simulink model "FullFMS_2026_02_18_V0_3_9"  (R2025b)
settings: Solver=ode23tb  StartTime=0.0  StopTime=inf  MaxStep=0.1  RelTol=1e-2
PreLoadFcn:
  | load("BUS_CONFIG.mat")
libraries: opcualib x8
(part 3 of 4)

== stateflow chart FullFMS_2026_02_18_V0_3_9/Chart ==
  state VarDeclaration_20
    entry:
    %Control_20
    C_24_CRoute_In  = Control_20.C_24_CRoute_In;
    C_25_CRoute_In  = Control_20.C_25_CRoute_In;
    C_26_CRoute_In  = Control_20.C_26_CRoute_In;
    C_27_CRoute_In  = Control_20.C_27_CRoute_In;
    C_28_CRoute_In  = Control_20.C_28_CRoute_In;
    C_29_CRoute_In  = Control_20.C_29_CRoute_In;
    C_24_Request    = Control_20.C_24_Request;
    C_24_CartDel    = Control_20.C_24_CartDel;
    C_24_CRoute_Out = Control_20.C_24_CRoute_Out;
    C_25_Request    = Control_20.C_25_Request;
    C_25_CartDel    = Control_20.C_25_CartDel;
    C_25_CRoute_Out = Control_20.C_25_CRoute_Out;
    C_26_Request    = Control_20.C_26_Request;
    C_26_CartDel    = Control_20.C_26_CartDel;
    C_26_CRoute_Out = Control_20.C_26_CRoute_Out;
    C_27_Request    = Control_20.C_27_Request;
    C_27_CartDel    = Control_20.C_27_CartDel;
    C_27_CRoute_Out = Control_20.C_27_CRoute_Out;
    C_28_Request    = Control_20.C_28_Request;
    C_28_CartDel    = Control_20.C_28_CartDel;
    C_28_CRoute_Out = Control_20.C_28_CRoute_Out;
    C_29_Request    = Control_20.C_29_Request;
    C_29_CartDel    = Control_20.C_29_CartDel;
    C_29_CRoute_Out = Control_20.C_29_CRoute_Out;
    %Actuators_20
    F_22_Led_On = Actuators_20.F_22_Led_On;
    F_22_Led_Off = Actuators_20.F_22_Led_Off;
    F_22_Conveyor = Actuators_20.F_22_Conveyor;
    F_24_Release_FB   = Actuators_20.F_24_Release_FB;
    F_25_Release_FB   = Actuators_20.F_25_Release_FB;
    F_26_Release_FB   = Actuators_20.F_26_Release_FB;
    F_27_Release_FB   = Actuators_20.F_27_Release_FB;
    F_28_Release_FB   = Actuators_20.F_28_Release_FB;
    F_29_Release_FB   = Actuators_20.F_29_Release_FB;
    %Sensors_20
    O_20_On            = Sensors_20.O_20_On;
    O_20_Off           = Sensors_20.O_20_Off;
    O_20_Controler_On  = Sensors_20.O_20_Controler_On;
    O_24_Cart_Stat     = Sensors_20.O_24_Cart_Stat;
    O_24_Cart_Next     = Sensors_20.O_24_Cart_Next;
    O_24_Optic         = Sensors_20.O_24_Optic;
    O_24_Count         = Sensors_20.O_24_Count;
    O_24_Pist_Bck      = Sensors_20.O_24_Pist_Bck;
    O_25_Cart_Stat     = Sensors_20.O_25_Cart_Stat;
    O_25_Cart_Next     = Sensors_20.O_25_Cart_Next;
    O_25_Optic         = Sensors_20.O_25_Optic;
    O_25_Count         = Sensors_20.O_25_Count;
    O_25_Pist_Back     = Sensors_20.O_25_Pist_Back;
    O_26_Cart_Stat     = Sensors_20.O_26_Cart_Stat;
    O_26_Cart_Next     = Sensors_20.O_26_Cart_Next;
    O_26_Optic         = Sensors_20.O_26_Optic;
    O_26_Count         = Sensors_20.O_26_Count;
    O_26_Pist_Back     = Sensors_20.O_26_Pist_Back;
    O_27_Cart_Stat     = Sensors_20.O_27_Cart_Stat;
    O_27_Cart_Next     = Sensors_20.O_27_Cart_Next;
    O_27_Optic         = Sensors_20.O_27_Optic;
    O_27_Count         = Sensors_20.O_27_Count;
    O_27_Pist_Back     = Sensors_20.O_27_Pist_Back;
    O_28_Cart_Stat     = Sensors_20.O_28_Cart_Stat;
    O_28_Cart_Next     = Sensors_20.O_28_Cart_Next;
    O_28_Optic         = Sensors_20.O_28_Optic;
    O_28_Count         = Sensors_20.O_28_Count;
    O_28_Pist_Back     = Sensors_20.O_28_Pist_Back;
    O_29_Cart_Stat     = Sensors_20.O_29_Cart_Stat;
    O_29_Cart_Next     = Sensors_20.O_29_Cart_Next;
    O_29_Optic         = Sensors_20.O_29_Optic;
    O_29_Count         = Sensors_20.O_29_Count;
    O_29_Pist_Back     = Sensors_20.O_29_Pist_Back;
  state VarDeclaration_30
    entry:
    %AS_i_30
    A_34_Request    = AS_i_30.A_34_Request;
    A_34_No_Cart    = AS_i_30.A_34_No_Cart;
    A_34_Cart_Full  = AS_i_30.A_34_Cart_Full;
    A_34_CRoute_Out = AS_i_30.A_34_CRoute_Out;
    A_32_RoboCartID = AS_i_30.A_32_RoboCartID;
    A_34_Cart_Stat  = AS_i_30.A_34_Cart_Stat;
    A_34_Cart_Next  = AS_i_30.A_34_Cart_Next;
    A_34_Optic      = AS_i_30.A_34_Optic;
    A_34_Count      = AS_i_30.A_34_Count;
    A_34_Pist_Bck   = AS_i_30.A_34_Pist_Bck;
    A_34_Release_FB = AS_i_30.A_34_Release_FB;
    A_34_CRoute_In  = AS_i_30.A_34_CRoute_in;
    %Control_30
    C_35_Part_Del = Control_30.C_35_Part_Del;
    C_30_Robot1   = Control_30.C_30_Robot1;
    C_30_Robot2   = Control_30.C_30_Robot2;
    %Actuators_30
    F_33_Led_Start  = Actuators_30.F_33_Led_Start;
    F_33_Led_Reset  = Actuators_30.F_33_Led_Reset;
    F_33_Led_Extra1 = Actuators_30.F_33_Led_Extra1;
    F_33_Led_Extra2 = Actuators_30.F_33_Led_Extra2;
    F_33_Spring_Cyl = Actuators_30.F_33_Spring_Cyl;
    F_33_Cover_Cyl  = Actuators_30.F_33_Cover_Cyl;
    %Sensors_30
    O_31_Start        = Sensors_30.O_31_Start;
    O_31_Stop         = Sensors_30.O_31_Stop;
    O_31_Reset        = Sensors_30.O_31_Reset;
    O_31_Part_in_Claw = Sensors_30.O_31_Part_in_Claw;
    O_31_Orientation  = Sensors_30.O_31_Orientation;
    O_32_Sp_Cyl_Bck   = Sensors_30.O_32_Sp_Cyl_Bck;
    O_32_Sp_Cyl_Fwd   = Sensors_30.O_32_Sp_Cyl_Fwd;
    O_32_Co_Cyl_Bck   = Sensors_30.O_32_Co_Cyl_Bck;
    O_32_Co_Cyl_Fwd   = Sensors_30.O_32_Co_Cyl_Fwd;
    O_32_Sp_PickUp    = Sensors_30.O_32_Sp_PickUp;
    O_32_Co_PickUp    = Sensors_30.O_32_Co_PickUp;
    O_32_CoMag_Empty  = Sensors_30.O_32_CoMag_Empty;
  state VarDeclaration_40
    entry:
    %AS_i_40
    A_44_Request = AS_i_40.A_44_Request;
    A_44_No_Cart = AS_i_40.A_44_No_Cart;
    A_44_Cart_Full = AS_i_40.A_44_Cart_Full;
    A_44_CRoute_In= AS_i_40.A_44_CRoute_In;
    A_43_StorCartID = AS_i_40.A_43_StorCartID;
    A_44_Cart_Stat = AS_i_40.A_44_Cart_Stat;
    A_44_Cart_Next = AS_i_40.A_44_Cart_Next;
    A_44_Optic = AS_i_40.A_44_Optic;
    A_44_Count =  AS_i_40.A_44_Count;
    A_44_Pist_Bck = AS_i_40.A_44_Pist_Bck;
    A_44_Release_FB = AS_i_40.A_44_Release_FB;
    A_44_CRoute_Out = AS_i_40.A_44_CRoute_Out;
    %Control_40
    C_45_Initialization = Control_40.C_45_Initialization;
    C_42_Profibus = Control_40.C_42_Profibus;
    C_45_Start = Control_40.C_45_Start;
    C_45_StorePart = Control_40.C_45_StorePart;
    C_45_RetrievePart = Control_40.C_45_RetrievePart;
    %Actuators_40
    F_43_Led_Start = Actuators_40.F_43_Led_Start;
    F_43_Led_Reset = Actuators_40.F_43_Led_Reset;
    F_43_Led_Extra1 = Actuators_40.F_43_Led_Extra1;
    F_43_Led_Extra2 = Actuators_40.F_43_Led_Extra2;
    F_43_Panel_O4 = Actuators_40.F_43_Panel_O4;
    F_43_Panel_O5 = Actuators_40.F_43_Panel_O5;
    F_43_Panel_O6 = Actuators_40.F_43_Panel_O6;
    F_43_Panel_O7 = Actuators_40.F_43_Panel_O7;
    %Sensors_40
    O_41_Start = Sensors_40.O_41_Start;
    O_41_Stop = Sensors_40.O_41_Stop;
    O_41_Key_Pos = Sensors_40.O_41_Key_Pos;
    O_41_Reset = Sensors_40.O_41_Reset;
    O_41_Panel_I4 = Sensors_40.O_41_Panel_I4;
    O_41_Panel_I5 = Sensors_40.O_41_Panel_I5;
    O_41_Panel_I6 = Sensors_40.O_41_Panel_I6;
    O_41_Panel_I7 = Sensors_40.O_41_Panel_I7;
  state VarDeclaration_50
    entry:
    %AS_i_50
    A_54_Request = AS_i_50.A_54_Request;
    A_54_No_Cart = AS_i_50.A_54_No_Cart;
    A_54_Cart_Full = AS_i_50.A_54_Cart_Full;
    A_54_CRoute_Out = AS_i_50.A_54_CRoute_Out;
    A_53_SortCartID = AS_i_50.A_53_SortCartID;
    A_54_Cart_Stat = AS_i_50.A_54_Cart_Stat;
    A_54_Cart_Next = AS_i_50.A_54_Cart_Next;
    A_54_Optic = AS_i_50.A_54_Optic;
    A_54_Count = AS_i_50.A_54_Count;
    A_54_Pist_Bck = AS_i_50.A_54_Pist_Bck;
    A_54_Release_FB = AS_i_50.A_54_Release_FB;
    A_54_CRoute_In = AS_i_50.A_54_CRoute_In;
    %Control_50
    C_55_Initialization = Control_50.C_55_Initialization;
    C_55_PD_Sort        = Control_50.C_55_PD_Sort;
    C_52_Profibus       = Control_50.C_52_Profibus;
    C_55_Start          = Control_50.C_55_Start;
    C_55_Cart2Del       = Control_50.C_55_Cart2Del;
    %Actuators_50
    F_52_Claw_2_Del  = Actuators_50.F_52_Claw_2_Del;
    F_52_Claw_2_Cart = Actuators_50.F_52_Claw_2_Cart;
    F_52_Claw_Down   = Actuators_50.F_52_Claw_Down;
    F_52_Close_Claw  = Actuators_50.F_52_Close_Claw;
    F_53_Led_Start   = Actuators_50.F_53_Led_Start;
    F_53_Led_Reset   = Actuators_50.F_53_Led_Reset;
    F_53_Led_Extra1  = Actuators_50.F_53_Led_Extra1;
    F_53_Led_Extra2  = Actuators_50.F_53_Led_Extra2;
    F_53_Panel_O4    = Actuators_50.F_53_Panel_O4;
    F_53_Panel_O5    = Actuators_50.F_53_Panel_O5;
    F_53_Panel_O6    = Actuators_50.F_53_Panel_O6;
    F_53_Panel_O7    = Actuators_50.F_53_Panel_O7;
    %Sensors_50
    O_50_Part_Reserve = Sensors_50.O_50_Part_Reserve;
    O_50_Claw_Cart    = Sensors_50.O_50_Claw_Cart;
    O_50_Claw_Del     = Sensors_50.O_50_Claw_Del;
    O_50_Claw_Reserve = Sensors_50.O_50_Claw_Reserve;
    O_50_Claw_Low     = Sensors_50.O_50_Claw_Low;
    O_50_Claw_High    = Sensors_50.O_50_Claw_High;
    O_50_Part_in_Claw = Sensors_50.O_50_Part_in_Claw;
    O_51_Start        = Sensors_50.O_51_Start;
    O_51_Stop         = Sensors_50.O_51_Stop;
    O_51_Key_Pos      = Sensors_50.O_51_Key_Pos;
    O_51_Reset        = Sensors_50.O_51_Reset;
    O_51_Panel_I4     = Sensors_50.O_51_Panel_I4;
    O_51_Panel_I5     = Sensors_50.O_51_Panel_I5;
    O_51_Panel_I6     = Sensors_50.O_51_Panel_I6;
    O_51_Panel_I7     = Sensors_50.O_51_Panel_I7;
  state VarDeclaration_60
    entry:
    %Control_60
    C_65_Initialization = Control_60.C_65_Initialization;
    C_65_ID_1    = Control_60.C_65_ID_1;
    C_65_ID_2    = Control_60.C_65_ID_2;
    C_62_Profibus    = Control_60.C_62_Profibus;
    C_65_RBS_Output    = Control_60.C_65_RBS_Output;
    C_65_RSB_Output    = Control_60.C_65_RSB_Output;
    C_65_BRS_Output    = Control_60.C_65_BRS_Output;
    C_65_BSR_Output    = Control_60.C_65_BSR_Output;
    C_65_SRB_Output    = Control_60.C_65_SRB_Output;
    C_65_SBR_Output    = Control_60.C_65_SBR_Output;
    %Actuators_60
    F_62_Conveyor  = Actuators_60.F_62_Conveyor;
    F_62_P1    = Actuators_60.F_62_P1;
    F_62_P2    = Actuators_60.F_62_P2;
    F_62_Identify  = Actuators_60.F_62_Identify;
    F_63_Led_Start  = Actuators_60.F_63_Led_Start;
    F_63_Led_Reset  = Actuators_60.F_63_Led_Reset;
    F_63_Led_Extra1 = Actuators_60.F_63_Led_Extra1;
    F_63_Led_Extra2 = Actuators_60.F_63_Led_Extra2;
    F_63_Panel_O4  = Actuators_60.F_63_Panel_O4;
    F_63_Panel_O5  = Actuators_60.F_63_Panel_O5;
    F_63_Panel_O6  = Actuators_60.F_63_Panel_O6;
    F_63_Panel_O7  = Actuators_60.F_63_Panel_O7;
    %Sensors_60
    O_60_SPart    = Sensors_60.O_60_SPart;
    O_60_Slnd    = Sensors_60.O_60_Slnd;
    O_60_SPhoto    = Sensors_60.O_60_SPhoto;
    O_60_Part_Pass  = Sensors_60.O_60_Part_Pass;
    O_60_SL1_Bck    = Sensors_60.O_60_SL1_Bck;
    O_60_SL1_Fwd    = Sensors_60.O_60_SL1_Fwd;
    O_60_SL2_Bck    = Sensors_60.O_60_SL2_Bck;
    O_60_SL2_Fwd    = Sensors_60.O_60_SL2_Fwd;
    O_61_Start    = Sensors_60.O_61_Start;
    O_61_Stop    = Sensors_60.O_61_Stop;
    O_61_Key_Pos    = Sensors_60.O_61_Key_Pos;
    O_61_Reset    = Sensors_60.O_61_Reset;
    O_61_Panel_I4  = Sensors_60.O_61_Panel_I4;
    O_61_Panel_I5  = Sensors_60.O_61_Panel_I5;
    O_61_Panel_I6  = Sensors_60.O_61_Panel_I6;
    O_61_Panel_I7  = Sensors_60.O_61_Panel_I7;
  state VarDeclaration_70
    entry:
    %AS_i_70
    A_74_Request = AS_i_70.A_74_Request;
    A_74_No_Cart = AS_i_70.A_74_No_Cart;
    A_74_Cart_Full = AS_i_70.A_74_Cart_Full;
    A_74_CRoute_Out = AS_i_70.A_74_CRoute_Out;
    A_74_CRoute_In80 = AS_i_70.A_74_CRoute_In80;
    A_73_TestCartID = AS_i_70.A_73_TestCartID;
    A_74_Cart_Stat = AS_i_70.A_74_Cart_Stat;
    A_74_Cart_Next = AS_i_70.A_74_Cart_Next;
    A_74_Optic = AS_i_70.A_74_Optic;
    A_74_Count = AS_i_70.A_74_Count;
    A_74_Pist_Bck = AS_i_70.A_74_Pist_Bck;
    A_74_Release_FB = AS_i_70.A_74_Release_FB;
    A_74_CRoute_In = AS_i_70.A_74_CRoute_In;
    %Control_70
    C_75_Initialization = Control_70.C_75_Initialization;
    C_75_ID_Delivery1 = Control_70.C_75_ID_Delivery1;
    C_75_ID_Delivery2 = Control_70.C_75_ID_Delivery2;
    C_75_Part_Del = Control_70.C_75_Part_Del;
    C_75_RQ_Part_Del = Control_70.C_75_RQ_Part_Del;
    C_75_RQ_Wrong = Control_70.C_75_RQ_Wrong;
    C_75_Identified80 = Control_70.C_75_Identified80;
    C_75_Requested80 = Control_70.C_75_Requested80;
    C_72_Profibus = Control_70.C_72_Profibus;
    C_75_RQ_Delivery1 = Control_70.C_75_RQ_Delivery1;
    C_75_RQ_Delivery2 = Control_70.C_75_RQ_Delivery2;
    C_75_Identified = Control_70.C_75_Identified;
    C_75_Requested = Control_70.C_75_Requested;
    %Actuators_70
    F_72_Elev_Down = Actuators_70.F_72_Elev_Down;
    F_72_Elev_Up = Actuators_70.F_72_Elev_Up;
    F_72_Eject_Part = Actuators_70.F_72_Eject_Part;
    F_72_Air_On = Actuators_70.F_72_Air_On;
    F_73_Led_Start = Actuators_70.F_73_Led_Start;
    F_73_Led_Reset = Actuators_70.F_73_Led_Reset;
    F_73_Led_Extra1 = Actuators_70.F_73_Led_Extra1;
    F_73_Led_Extra2 = Actuators_70.F_73_Led_Extra2;
    F_73_Panel_O4 = Actuators_70.F_73_Panel_O4;
    F_73_Panel_O5 = Actuators_70.F_73_Panel_O5;
    F_73_Panel_O6 = Actuators_70.F_73_Panel_O6;
    F_73_Panel_O7 = Actuators_70.F_73_Panel_O7;
    %Sensors_70
    O_70_SInductive = Sensors_70.O_70_SInductive;
    O_70_SPart = Sensors_70.O_70_SPart;
    O_70_SStation = Sensors_70.O_70_SStation;
    O_70_SPart_Height = Sensors_70.O_70_SPart_Height;
    O_70_Elev_High = Sensors_70.O_70_Elev_High;
    O_70_Elev_Low = Sensors_70.O_70_Elev_Low;
    O_70_Pist_Back = Sensors_70.O_70_Pist_Back;
    O_71_Start = Sensors_70.O_71_Start;
    O_71_Stop = Sensors_70.O_71_Stop;
    O_71_Key_Pos = Sensors_70.O_71_Key_Pos;
    O_71_Reset = Sensors_70.O_71_Reset;
    O_71_Panel_I4 = Sensors_70.O_71_Panel_I4;
    O_71_Panel_I5 = Sensors_70.O_71_Panel_I5;
    O_71_Panel_I6 = Sensors_70.O_71_Panel_I6;
    O_71_Panel_I7 = Sensors_70.O_71_Panel_I7;
  state VarDeclaration_80
    entry:
    %Control_80
    C_85_Initialization = Control_80.C_85_Initialization;
    C_85_Part_Del = Control_80.C_85_Part_Del;
    C_85_Part_Mag = Control_80.C_85_Part_Mag;
    C_86_Mag_Parts = Control_80.C_86_Mag_Parts;
    C_87_RQ_MParts = Control_80.C_87_RQ_MParts;
    C_82_Profibus = Control_80.C_82_Profibus;
    C_83_RQ_Parts = Control_80.C_83_RQ_Parts;
    C_85_Start = Control_80.C_85_Start;
    C_85_Single = Control_80.C_85_Single;
    C_85_Continuous = Control_80.C_85_Continuous;
    C_85_Counted = Control_80.C_85_Counted;
    %Actuators_80
    F_82_Pist_Adv = Actuators_80.F_82_Pist_Adv;
    F_82_Suction_On = Actuators_80.F_82_Suction_On;
    F_82_Suction_Off = Actuators_80.F_82_Suction_Off;
    F_82_Arm_2_Del = Actuators_80.F_82_Arm_2_Del;
    F_82_Arm_2_Mag = Actuators_80.F_82_Arm_2_Mag;
    F_83_Led_Start = Actuators_80.F_83_Led_Start;
    F_83_Led_Reset = Actuators_80.F_83_Led_Reset;
    F_83_Led_Extra1 = Actuators_80.F_83_Led_Extra1;
    F_83_Led_Extra2 = Actuators_80.F_83_Led_Extra2;
    F_83_Panel_O4 = Actuators_80.F_83_Panel_O4;
    F_83_Panel_O5 = Actuators_80.F_83_Panel_O5;
    F_83_Panel_O6 = Actuators_80.F_83_Panel_O6;
    F_83_Panel_O7 = Actuators_80.F_83_Panel_O7;
    %Sensors_80
    O_80_Mag_Full = Sensors_80.O_80_Mag_Full;
    O_80_Pist_Back = Sensors_80.O_80_Pist_Back;
    O_80_Pist_Fwd = Sensors_80.O_80_Pist_Fwd;
    O_80_Part_Stuck = Sensors_80.O_80_Part_Stuck;
    O_80_Arm_Mag = Sensors_80.O_80_Arm_Mag;
    O_80_Arm_Del = Sensors_80.O_80_Arm_Del;
    O_80_Mag_Empty = Sensors_80.O_80_Mag_Empty;
    O_81_Start = Sensors_80.O_81_Start;
    O_81_Stop = Sensors_80.O_81_Stop;
    O_81_Key_Pos = Sensors_80.O_81_Key_Pos;
    O_81_Reset = Sensors_80.O_81_Reset;
    O_81_Panel_I4 = Sensors_80.O_81_Panel_I4;
    O_81_Panel_I5 = Sensors_80.O_81_Panel_I5;
    O_81_Panel_I6 = Sensors_80.O_81_Panel_I6;
    O_81_Panel_I7 = Sensors_80.O_81_Panel_I7;
  state VarDeclaration_90
    entry:
    %AS_i_90
    A_94_Request    = AS_i_90.A_94_Request;
    A_94_No_Cart    = AS_i_90.A_94_No_Cart;
    A_94_Cart_Full  = AS_i_90.A_94_Cart_Full;
    A_94_CRoute_Out = AS_i_90.A_94_CRoute_Out;
    A_93_ProcCartID = AS_i_90.A_93_ProcCartID;
    A_94_Cart_Stat  = AS_i_90.A_94_Cart_Stat;
    A_94_Cart_Next  = AS_i_90.A_94_Cart_Next;
    A_94_Optic      = AS_i_90.A_94_Optic;
    A_94_Count      = AS_i_90.A_94_Count;
    A_94_Pist_Bck   = AS_i_90.A_94_Pist_Bck;
    A_94_Release_FB = AS_i_90.A_94_Release_FB;
    A_94_CRoute_In  = AS_i_90.A_94_CRoute_In;
    %Control_90
    C_95_Initialization = Control_90.C_95_Initialization;
    C_95_PD_Proc        = Control_90.C_95_PD_Proc;
    C_95_PD_Cart        = Control_90.C_95_PD_Cart;
    C_92_Profibus       = Control_90.C_92_Profibus;
    C_95_Start          = Control_90.C_95_Start
    C_95_Cart2Del       = Control_90.C_95_Cart2Del;
    C_95_Del2Cart       = Control_90.C_95_Del2Cart;
    %Actuators_90
    F_92_Claw_2_Cart = Actuators_90.F_92_Claw_2_Cart;
    F_92_Claw_2_Del = Actuators_90.F_92_Claw_2_Del;
    F_92_Claw_Down = Actuators_90.F_92_Claw_Down;
    F_92_Close_Claw = Actuators_90.F_92_Close_Claw;
    F_93_Led_Start = Actuators_90.F_93_Led_Start;
    F_93_Led_Reset = Actuators_90.F_93_Led_Reset;
    F_93_Led_Extra1 = Actuators_90.F_93_Led_Extra1;
    F_93_Led_Extra2 = Actuators_90.F_93_Led_Extra2;
    F_93_Panel_O4 = Actuators_90.F_93_Panel_O4;
    F_93_Panel_O5 = Actuators_90.F_93_Panel_O5;
    F_93_Panel_O6 = Actuators_90.F_93_Panel_O6;
    F_93_Panel_O7 = Actuators_90.F_93_Panel_O7;
    %Sensors_90
    O_90_Part_Reserve = Sensors_90.O_90_Part_Reserve;
    O_90_Claw_Del = Sensors_90.O_90_Claw_Del;
    O_90_Claw_Cart = Sensors_90.O_90_Claw_Cart;
    O_90_Claw_Reserve = Sensors_90.O_90_Claw_Reserve;
    O_90_Claw_Low = Sensors_90.O_90_Claw_Low;
    O_90_Claw_High = Sensors_90.O_90_Claw_High;
    O_90_Part_in_Claw = Sensors_90.O_90_Part_in_Claw;
    O_91_Start = Sensors_90.O_91_Start;
    O_91_Stop = Sensors_90.O_91_Stop;
    O_91_Key_Pos = Sensors_90.O_91_Key_Pos;
    O_91_Reset = Sensors_90.O_91_Reset;
    O_91_Panel_I4 = Sensors_90.O_91_Panel_I4;
    O_91_Panel_I5 = Sensors_90.O_91_Panel_I5;
    O_91_Panel_I6 = Sensors_90.O_91_Panel_I6;
    O_91_Panel_I7 = Sensors_90.O_91_Panel_I7;
  state VarDeclaration_100
    entry:
    %Control_100
    C_105_Initialization = Control_100.C_105_Initialization;
    C_105_Part_ready     = Control_100.C_105_Part_ready;
    C_105_Test_Ok        = Control_100.C_105_Test_Ok;
    C_105_Test_Fail      = Control_100.C_105_Test_Fail;
    C_102_Profibus       = Control_100.C_102_Profibus;
    C_103_RQ_Turns       = Control_100.C_103_RQ_Turns;
    C_105_Start          = Control_100.C_105_Start;
    C_105_Test           = Control_100.C_105_Test;
    C_105_TestDrill      = Control_100.C_105_TestDrill;
    C_105_Rotation       = Control_100.C_105_Rotation;
    %Actuators_100
    F_102_Drill_On   = Actuators_100.F_102_Drill_On;
    F_102_RT_On      = Actuators_100.F_102_RT_On;
    F_102_Drill_Down = Actuators_100.F_102_Drill_Down;
    F_102_Drill_Up   = Actuators_100.F_102_Drill_Up;
    F_102_Drill_Pin  = Actuators_100.F_102_Drill_Pin;
    F_102_Test_Pin   = Actuators_100.F_102_Test_Pin;
    F_103_Led_Start  = Actuators_100.F_103_Led_Start;
    F_103_Led_Reset  = Actuators_100.F_103_Led_Reset;
    F_103_Led_Extra1 = Actuators_100.F_103_Led_Extra1;
    F_103_Led_Extra2 = Actuators_100.F_103_Led_Extra2;
    F_103_Panel_O4   = Actuators_100.F_103_Panel_O4;
    F_103_Panel_O5   = Actuators_100.F_103_Panel_O5;
    F_103_Panel_O6   = Actuators_100.F_103_Panel_O6;
    F_103_Panel_O7   = Actuators_100.F_103_Panel_O7
    %Sensors_100
    O_100_PInit_Pos   = Sensors_100.O_100_PInit_Pos;
    O_100_PDrill_Pos  = Sensors_100.O_100_PDrill_Pos;
    O_100_PTest_Pos   = Sensors_100.O_100_PTest_Pos;
    O_100_SDrill_High = Sensors_100.O_100_SDrill_High;
    O_100_SDrill_Low  = Sensors_100.O_100_SDrill_Low;
    O_100_RT_Sensor   = Sensors_100.O_100_RT_Sensor;
    O_100_PTest_Ok    = Sensors_100.O_100_PTest_Ok;
    O_101_Start       = Sensors_100.O_101_Start;
    O_101_Stop        = Sensors_100.O_101_Stop;
    O_101_Key_Pos     = Sensors_100.O_101_Key_Pos;
    O_101_Reset       = Sensors_100.O_101_Reset;
    O_101_Panel_I4    = Sensors_100.O_101_Panel_I4;
    O_101_Panel_I5    = Sensors_100.O_101_Panel_I5;
    O_101_Panel_I6    = Sensors_100.O_101_Panel_I6;
    O_101_Panel_I7    = Sensors_100.O_101_Panel_I7;
  state Start
    during:
    Control_20.C_24_Request
  state CartToTesting
    state InitialCondition
      entry:
      status = false;
      during:
      Control_20.C_24_Request
      Actuators_20.F_22_Conveyor
      Actuators_20.F_29_Release_FB
      AS_i_50.A_54_Release_FB
      AS_i_50.A_53_SortCartID
      Sensors_20.O_29_Pist_Back
      AS_i_50.A_54_Pist_Bck
      Sensors_20.O_29_Cart_Stat
      AS_i_50.A_54_Cart_Stat
      AS_i_50.A_54_No_Cart
      Actuators_50.F_53_Led_Extra1
      Sensors_20.O_29_Cart_Next
      AS_i_50.A_54_Cart_Next
      AS_i_70.A_73_TestCartID
      Sensors_20.O_24_Cart_Stat
      AS_i_70.A_74_Cart_Stat
      Control_20.C_24_CartDel
      AS_i_70.A_74_No_Cart
      Actuators_70.F_73_Led_Extra1
      AS_i_70.A_74_CRoute_In
      if ~Control_20.C_24_Request && ...
      ~Actuators_20.F_22_Conveyor && ...
      ~Actuators_20.F_29_Release_FB && ...
      ~AS_i_50.A_54_Release_FB && ...
      AS_i_50.A_53_SortCartID ~= 0 && ...
      ~Sensors_20.O_29_Pist_Back && ...
      ~AS_i_50.A_54_Pist_Bck && ...
      Sensors_20.O_29_Cart_Stat && ...
      AS_i_50.A_54_Cart_Stat && ...
      ~AS_i_50.A_54_No_Cart && ...
      ~Actuators_50.F_53_Led_Extra1 && ...
      ~Sensors_20.O_29_Cart_Next && ...
      ~AS_i_50.A_54_Cart_Next && ...
      AS_i_70.A_73_TestCartID == 0 && ...
      ~Sensors_20.O_24_Cart_Stat && ...
      ~AS_i_70.A_74_Cart_Stat && ...
      ~Control_20.C_24_CartDel && ...
      AS_i_70.A_74_No_Cart && ...
      Actuators_70.F_73_Led_Extra1 && ...
      ~AS_i_70.A_74_CRoute_In
      status = true;
      else
      status = false;
      end
    state StartsProcess
      entry:
      status2 = false;
      during:
      Control_20.C_24_Request;
      Actuators_20.F_22_Conveyor;
      Actuators_20.F_29_Release_FB;
      AS_i_50.A_54_Release_FB;
      AS_i_50.A_53_SortCartID;
      Sensors_20.O_29_Pist_Back;
      AS_i_50.A_54_Pist_Bck;
      if Control_20.C_24_Request && ...
      Actuators_20.F_22_Conveyor && ...
      Actuators_20.F_29_Release_FB && ...
      AS_i_50.A_54_Release_FB && ...
      AS_i_50.A_53_SortCartID == 0 && ...
      Sensors_20.O_29_Pist_Back && ...
      AS_i_50.A_54_Pist_Bck
      status2 = true;
      else
      status2 = false;
      end
    state CartStartsMoving
      entry:
      status3 = false;
      during:
      Sensors_20.O_29_Cart_Stat
      AS_i_50.A_54_Cart_Stat
      AS_i_50.A_54_No_Cart
      Actuators_50.F_53_Led_Extra1
      if ~Sensors_20.O_29_Cart_Stat && ...
      ~AS_i_50.A_54_Cart_Stat && ...
      AS_i_50.A_54_No_Cart && ...
      Actuators_50.F_53_Led_Extra1
      status3 = true;
      else
      status3 = false;
      end
    state CartGetsNearNextStation
      entry:
      status4 = false;
      during:
      Actuators_20.F_29_Release_FB
      AS_i_50.A_54_Release_FB
      Sensors_20.O_29_Pist_Back
      AS_i_50.A_54_Pist_Bck
      Sensors_20.O_29_Cart_Next
      AS_i_50.A_54_Cart_Next
      if ~Actuators_20.F_29_Release_FB && ...
      ~AS_i_50.A_54_Release_FB && ...
      ~Sensors_20.O_29_Pist_Back && ...
      ~AS_i_50.A_54_Pist_Bck && ...
      Sensors_20.O_29_Cart_Next && ...
      AS_i_50.A_54_Cart_Next
      status4 = true;
      else
      status4 = false;
      end
    state DetectionofCartNumberinStation
      entry:
      status5 = false;
      during:
      AS_i_70.A_73_TestCartID
      if ~AS_i_70.A_73_TestCartID
      status5 = true;
      end
    state CartPassesNextStation
      entry:
      status6 = false;
      during:
      Sensors_20.O_29_Cart_Next
      AS_i_50.A_54_Cart_Next
      if ~Sensors_20.O_29_Cart_Next && ...
      ~AS_i_50.A_54_Cart_Next
      status6 = true;
      else
      status6 = false;
      end
    state CartArrivesinNextStation
      entry:
      status7 = false;
      during:
      Sensors_20.O_24_Cart_Stat
      AS_i_70.A_74_Cart_Stat
      Control_20.C_24_CartDel
      AS_i_70.A_74_No_Cart
      Actuators_70.F_73_Led_Extra1
      AS_i_70.A_74_CRoute_In
      if Sensors_20.O_24_Cart_Stat &&...
      AS_i_70.A_74_Cart_Stat &&...
      Control_20.C_24_CartDel &&...
      ~AS_i_70.A_74_No_Cart &&...
      ~Actuators_70.F_73_Led_Extra1 &&...
      AS_i_70.A_74_CRoute_In
      status7 = true;
      else
      status7 = false;
      end
    state T3
      during:
      Control_20.C_24_CartDel
    state T2
      during:
      AS_i_70.A_74_CRoute_In
    state T1
      during:
      Control_20.C_24_Request
    (default) -> CartToTesting.InitialCondition
    CartToTesting.CartStartsMoving -> CartToTesting.CartGetsNearNextStation : [Sensors_20.O_29_Cart_Next == true && ...
        | status3 == true]
    CartToTesting.DetectionofCartNumberinStation -> CartToTesting.CartPassesNextStation : [Sensors_20.O_29_Cart_Next == false && ...
        | status5 == true]
    CartToTesting.CartGetsNearNextStation -> CartToTesting.DetectionofCartNumberinStation : [AS_i_70.A_73_TestCartID == 0 && ...
        | status4 == true]
    CartToTesting.CartPassesNextStation -> CartToTesting.CartArrivesinNextStation : [Sensors_20.O_24_Cart_Stat == true && ...
        | status6 == true]
    CartToTesting.StartsProcess -> CartToTesting.CartStartsMoving [order 1] : [Sensors_20.O_29_Cart_Stat == false && ...
        |  status2 == true]
    CartToTesting.InitialCondition -> CartToTesting.StartsProcess : [Control_20.C_24_Request == true && ...
        |  status == true]
    CartToTesting.CartArrivesinNextStation -> (junction 582)
    CartToTesting.StartsProcess -> CartToTesting.T1 [order 2] : [after(2, sec)]
    (junction 582) -> CartToTesting.T3 [order 2] : [after(3,sec)]
    (junction 582) -> CartToTesting.T2 [order 1] : [after(2,sec)]
  state Distribution_Single
    state InitialCondition
      entry:
      status = false;
      during:
      Sensors_70.O_70_SStation
      Control_70.C_75_RQ_Wrong
      AS_i_70.A_74_CRoute_In80
      Control_80.C_85_Single
      Control_80.C_85_Start
      Control_80.C_85_Part_Del
      Control_80.C_86_Mag_Parts
      Actuators_80.F_82_Pist_Adv
      Actuators_80.F_82_Arm_2_Del
      Actuators_80.F_82_Arm_2_Mag
      Actuators_80.F_82_Suction_On
      Actuators_80.F_82_Suction_Off
      Actuators_80.F_83_Led_Extra1
      Sensors_80.O_80_Arm_Mag
      Sensors_80.O_80_Arm_Del
      Sensors_80.O_80_Pist_Back
      Sensors_80.O_80_Pist_Fwd
      Sensors_80.O_80_Part_Stuck
      Sensors_80.O_81_Start
      Sensors_80.O_81_Key_Pos
      if ~Sensors_70.O_70_SStation && ...
      ~Control_70.C_75_RQ_Wrong && ...
      ~AS_i_70.A_74_CRoute_In80 && ...
      Control_80.C_85_Single && ...
      ~Control_80.C_85_Start && ...
      ~Control_80.C_85_Part_Del && ...
      Control_80.C_86_Mag_Parts ~= 0 && ...
      ~Actuators_80.F_82_Pist_Adv && ...
      ~Actuators_80.F_82_Arm_2_Del && ...
      ~Actuators_80.F_82_Arm_2_Mag && ...
      ~Actuators_80.F_82_Suction_On && ...
      ~Actuators_80.F_82_Suction_Off && ...
      ~Actuators_80.F_83_Led_Extra1 && ...
      Sensors_80.O_80_Arm_Mag && ...
      ~Sensors_80.O_80_Arm_Del && ...
      Sensors_80.O_80_Pist_Back && ...
      ~Sensors_80.O_80_Pist_Fwd && ...
      ~Sensors_80.O_80_Part_Stuck && ...
      ~Sensors_80.O_81_Start && ...
      Sensors_80.O_81_Key_Pos
      status = true;
      else
      status = false;
      end
    state ArmToDelivery
      entry:
      status1 = false;
      during:
      Actuators_80.F_82_Arm_2_Del
      if Actuators_80.F_82_Arm_2_Del
      status1 = true;
      else
      status1 = false;
      end
    state ArmArrives_FeedsPart
      entry:
      status3 = false;
      during:
      Actuators_80.F_82_Pist_Adv
      Actuators_80.F_82_Arm_2_Del
      Sensors_80.O_80_Arm_Del
      if Actuators_80.F_82_Pist_Adv && ...
      ~Actuators_80.F_82_Arm_2_Del && ...
      Sensors_80.O_80_Arm_Del
      status3 = true;
      else
      status3 = false;
      end
    state PartFed
      entry:
      status5 = false;
      during:
      Control_80.C_86_Mag_Parts
      Actuators_80.F_82_Pist_Adv
      Sensors_80.O_80_Pist_Fwd
      if Control_80.C_86_Mag_Parts ~= 0 && ...
      ~Actuators_80.F_82_Pist_Adv && ...
      Sensors_80.O_80_Pist_Fwd
      status5 = true;
      else
      status5 = false;
      end
    state ArmToMagazine
      entry:
      status7 = false;
      during:
      Actuators_80.F_82_Arm_2_Mag
      if Actuators_80.F_82_Arm_2_Mag
      status7 = true;
      else
      status7 = false;
      end
    state ArmArrives_PicksPart
      entry:
      status9 = false;
      during:
      Actuators_80.F_82_Arm_2_Mag
      Actuators_80.F_82_Suction_On
      if ~Actuators_80.F_82_Arm_2_Mag && ...
      Actuators_80.F_82_Suction_On
      status9 = true;
      else
      status9 = false;
      end
    state ArmToDelivery1
      entry:
      status10 = false;
      during:
      Actuators_80.F_82_Arm_2_Del
      if Actuators_80.F_82_Arm_2_Del
      status10 = true;
      else
      status10 = false;
      end
    state ArmArrives_DeliversPart
      entry:
      status12 = false;
      during:
      Actuators_80.F_82_Arm_2_Del
      Actuators_80.F_82_Suction_On
      Actuators_80.F_82_Suction_Off
      if ~Actuators_80.F_82_Arm_2_Del && ...
      ~Actuators_80.F_82_Suction_On && ...
      Actuators_80.F_82_Suction_Off
      status12 = true;
      else
      status12 = false;
      end
    state ArmToMagazine1
      entry:
      status13 = false;
      during:
      Control_80.C_85_Part_Del
      Actuators_80.F_82_Arm_2_Mag
      Actuators_80.F_82_Suction_Off
      Actuators_80.F_83_Led_Extra1
      if Control_80.C_85_Part_Del && ...
      ~Actuators_80.F_82_Arm_2_Mag && ...
      ~Actuators_80.F_82_Suction_Off && ...
      Actuators_80.F_83_Led_Extra1
      status13 = true;
      else
      status13 = false;
      end
    state ArmArrives_Finish
      during:
      Actuators_80.F_82_Arm_2_Mag
    state ArmCloseDelivery
      entry:
      status2 = false;
      during:
      Sensors_70.O_70_SStation
      if Sensors_70.O_70_SStation
      status2 = true;
      else
      status2 = false;
      end
    state PistonStartsMoveForward
      entry:
      status4 = false;
      during:
      Sensors_80.O_80_Pist_Back
      if ~Sensors_80.O_80_Pist_Back
      status4 = true;
      else
      status4 = false;
      end
    state PistonStartsMoveBackward
      entry:
      status6 = false;
      during:
      Sensors_80.O_80_Pist_Fwd
      if ~Sensors_80.O_80_Pist_Fwd
      status6 = true;
      else
      status6 = false;
      end
    state ArmCloseDeliver1
      entry:
      status8 = false;
      during:
      Sensors_70.O_70_SStation
      if ~Sensors_70.O_70_SStation
      status8 = true;
      else
      status8 = false;
      end
    state ArmCloseDelivery2
      entry:
      status11 = false;
      during:
      Sensors_70.O_70_SStation
      if Sensors_70.O_70_SStation
      status11 = true;
      else
      status11 = false;
      end
    state ArmCloseDeliver3
      entry:
      status14 = false;
      during:
      Sensors_70.O_70_SStation
      if ~Sensors_70.O_70_SStation
      status14 = true;
      else
      status14 = false;
      end
    state T1
      during:
      Control_80.C_85_Part_Del
      Actuators_80.F_83_Led_Extra1
    (default) -> Distribution_Single.InitialCondition
    Distribution_Single.ArmArrives_DeliversPart -> Distribution_Single.ArmToMagazine1 : [Sensors_80.O_80_Part_Stuck == false && ...
        | status12 == true]
    Distribution_Single.ArmToMagazine -> Distribution_Single.ArmArrives_PicksPart [order 2] : [Sensors_80.O_80_Arm_Mag == true && ...
        | status8 == true]
    Distribution_Single.ArmToDelivery1 -> Distribution_Single.ArmArrives_DeliversPart [order 2] : [Sensors_80.O_80_Arm_Del == true && ...
        | status11 == true]
    Distribution_Single.ArmToDelivery -> Distribution_Single.ArmArrives_FeedsPart [order 2] : [Sensors_80.O_80_Arm_Del == true && ...
        | status2 == true]
    Distribution_Single.ArmArrives_PicksPart -> Distribution_Single.ArmToDelivery1 : [Sensors_80.O_80_Part_Stuck == true && ...
        | status9 == true]
    Distribution_Single.ArmToMagazine1 -> Distribution_Single.ArmArrives_Finish [order 2] : [Sensors_80.O_80_Arm_Mag == true && ...
        | status14 == true]
    Distribution_Single.ArmArrives_FeedsPart -> Distribution_Single.PartFed [order 2] : [Sensors_80.O_80_Pist_Fwd == true && ...
        | status4 == true]
    Distribution_Single.PartFed -> Distribution_Single.ArmToMagazine [order 2] : [Sensors_80.O_80_Pist_Back == true && ...
        | status6 == true]
    Distribution_Single.InitialCondition -> Distribution_Single.ArmToDelivery : [Sensors_80.O_81_Start == true | ...
        | Control_80.C_85_Start == true | ...
        | Control_70.C_75_RQ_Wrong == true | ...
        | (AS_i_70.A_74_CRoute_In80 == true && Sensors_80.O_81_Key_Pos == true) ]
    Distribution_Single.ArmToDelivery -> Distribution_Single.ArmCloseDelivery [order 1] : [Sensors_80.O_80_Arm_Mag == false &&...
        |  status1 == true]
    Distribution_Single.ArmToDelivery1 -> Distribution_Single.ArmCloseDelivery2 [order 1] : [Sensors_80.O_80_Arm_Mag == false &&...
        |  status10 == true]
    Distribution_Single.ArmToMagazine -> Distribution_Single.ArmCloseDeliver1 [order 1] : [Sensors_80.O_80_Arm_Del == false &&...
        |  status7 == true]
    Distribution_Single.ArmArrives_FeedsPart -> Distribution_Single.PistonStartsMoveForward [order 1] : [status3 == true]
    Distribution_Single.PartFed -> Distribution_Single.PistonStartsMoveBackward [order 1] : [status5 == true]
    Distribution_Single.ArmToMagazine1 -> (junction 650) [order 1]
    (junction 650) -> ArmCloseDeliver3 [order 1] : [Sensors_80.O_80_Arm_Del == false &&...
        |  status13 == true]
    (junction 650) -> Distribution_Single.T1 [order 2] : after(4,sec)
  state Identified_Delivery
    state InitialCondition
      entry:
      status = false;
      during:
      AS_i_70.A_74_Cart_Full;
      AS_i_70.A_74_CRoute_Out;
      AS_i_70.A_74_Optic;
      Control_70.C_75_ID_Delivery1;
      Control_70.C_75_ID_Delivery2;
      Control_70.C_75_Part_Del;
      Control_70.C_75_Identified;
      Actuators_70.F_72_Elev_Down;
      Actuators_70.F_72_Elev_Up;
      Actuators_70.F_72_Eject_Part;
      Actuators_70.F_72_Air_On;
      Actuators_70.F_73_Led_Extra1;
      Actuators_70.F_73_Led_Extra2;
      Sensors_70.O_70_SInductive;
      Sensors_70.O_70_SPart;
      Sensors_70.O_70_SStation;
      Sensors_70.O_70_SPart_Height;
      Sensors_70.O_70_Elev_High;
      Sensors_70.O_70_Elev_Low;
      Sensors_70.O_70_Pist_Back;
      Sensors_70.O_71_Start;
      Sensors_70.O_71_Stop;
      Sensors_70.O_71_Key_Pos;
      Sensors_70.O_71_Reset;
      Sensors_80.O_80_Arm_Mag
      if Control_70.C_75_Identified && ...
      ~Sensors_70.O_70_SPart && ...
      ~Sensors_80.O_80_Arm_Mag
      status = true;
      else
      status = false;
      end
    state Part_Arrives
      entry:
      status1 = false;
      MetalicPart = false;
      during:
      Control_70.C_75_ID_Delivery2;
      Sensors_70.O_70_SInductive;
      Sensors_70.O_70_SPart;
      Sensors_80.O_80_Arm_Mag
      if Sensors_70.O_70_SInductive
      MetalicPart = true
      else
      MetalicPart = false
      end
      if Sensors_70.O_70_SPart && ...
      ((Sensors_70.O_70_SInductive && ...
      Control_70.C_75_ID_Delivery2) | ...
      (~Sensors_70.O_70_SInductive && ...
      ~Control_70.C_75_ID_Delivery2)) && ...
      ~Sensors_80.O_80_Arm_Mag
      status1 = true;
      else
      status1 =false;
      end
    state Elevator_Up
      entry:
      status2 = false;
      during:
      Actuators_70.F_72_Elev_Up;
      if Actuators_70.F_72_Elev_Up
      status2 = true
      else
      status2 = false
      end
    state Elevator_StartsMovingUp
      entry:
      status3 = false;
      during:
      Sensors_70.O_70_SInductive;
      if ~Sensors_70.O_70_SInductive
      status3 = true
      else
      status3 = false
      end
    state Elevator_MiddleUp
      entry:
      status4 = false;
      during:
      Sensors_70.O_70_SStation;
      if ~Sensors_70.O_70_SStation
      status4 = true
      else
      status4 = false
      end
    state Elevator_High
      entry:
      status5 = false;
      during:
      MetalicPart;
      Control_70.C_75_ID_Delivery1;
      Control_70.C_75_ID_Delivery2;
      Sensors_70.O_70_SPart_Height;
      if MetalicPart && ...
      Control_70.C_75_ID_Delivery2 && ...
      ~Control_70.C_75_ID_Delivery1;
      status5 = true
      end
      if ~MetalicPart && ...
      Control_70.C_75_ID_Delivery1 && ...
      ((Sensors_70.O_70_SPart_Height && ...
      Control_70.C_75_ID_Delivery2) | ...
      (~Sensors_70.O_70_SPart_Height && ...
      ~Control_70.C_75_ID_Delivery2))
      status5=true
      end
    state Part_HeightSensor
      entry:
      status7 = false;
      during:
      Actuators_70.F_72_Eject_Part;
      Sensors_70.O_70_Pist_Back;
      Sensors_70.O_70_SPart_Height
      if Actuators_70.F_72_Eject_Part && ...
      ~Sensors_70.O_70_Pist_Back && ...
      ~Sensors_70.O_70_SPart_Height
      status7 = true
      else
      status7 = false
      end
    state Piston_Back
      entry:
      status8 = false;
      during:
      Actuators_70.F_72_Eject_Part
      if ~Actuators_70.F_72_Eject_Part
      status8 = true
      else
      status8 = false
      end
    state Elevator_StartsMovingDown
      entry:
      status10 = false;
      during:
      Actuators_70.F_72_Elev_Down;
      Actuators_70.F_72_Elev_Up;
      if Actuators_70.F_72_Elev_Down && ...
      ~Actuators_70.F_72_Elev_Up
      status10 = true
      else
      status10 = false
      end
    state Elevator_MiddleDown
      entry:
      status11 = false;
      during:
      Sensors_70.O_70_SStation;
      if ~Sensors_70.O_70_SStation
      status11 = true
      else
      status11 = false
      end
    state Elevator_InductiveDown
      entry:
      status12 = false;
      during:
      Sensors_70.O_70_SInductive;
      if ~Sensors_70.O_70_SInductive
      status12 = true
      else
      status12 = false
      end
    state Elevator_Down
      entry:
      status13 = false;
      during:
      AS_i_70.A_74_CRoute_Out;
      Actuators_70.F_72_Elev_Down;
      Control_70.C_75_Part_Del;
      if AS_i_70.A_74_CRoute_Out && ...
      ~Actuators_70.F_72_Elev_Down&& ...
      Control_70.C_75_Part_Del
      status13 = true
      else
      status13 = false
      end
    state Pushes_Part
      entry:
      status6 = false;
      during:
      Actuators_70.F_72_Eject_Part;
      Actuators_70.F_72_Air_On;
      Sensors_70.O_70_SPart
      if Actuators_70.F_72_Eject_Part && ...
      Actuators_70.F_72_Air_On && ...
      ~Sensors_70.O_70_SStation
      status6 = true
      else
      status6 = false
      end
    state Part_ArrivesAtCart
      entry:
      status9 = false;
      during:
      AS_i_70.A_74_Cart_Full;
      AS_i_70.A_74_Optic;
      Actuators_70.F_72_Air_On;
      Actuators_70.F_73_Led_Extra2
      if AS_i_70.A_74_Optic && ...
      AS_i_70.A_74_Cart_Full && ...
      ~Actuators_70.F_72_Air_On && ...
      Actuators_70.F_73_Led_Extra2;
      status9 = true
      else
      status9 = false
      end
    state End_Process
      entry:
      status14 = false;
      during:
      AS_i_70.A_74_CRoute_Out;
      if  ~AS_i_70.A_74_CRoute_Out;
      status14 = true
      else
      status14 = false
      end
    (default) -> Identified_Delivery.InitialCondition
    Identified_Delivery.Part_HeightSensor -> Identified_Delivery.Piston_Back [order 1] : after (2,sec)
    Identified_Delivery.Elevator_StartsMovingDown -> Identified_Delivery.Elevator_MiddleDown : [status10 == true && Sensors_70.O_70_SStation == true]
    Identified_Delivery.Elevator_StartsMovingUp -> Identified_Delivery.Elevator_MiddleUp : [status3 == true && Sensors_70.O_70_SStation == true]
    Identified_Delivery.Elevator_MiddleUp -> Identified_Delivery.Elevator_High : [status4 == true && Sensors_70.O_70_Elev_High == true]
    Identified_Delivery.Elevator_Up -> Identified_Delivery.Elevator_StartsMovingUp : [status2 == true && Sensors_70.O_70_SInductive == true ]
    Identified_Delivery.Piston_Back -> Identified_Delivery.Elevator_StartsMovingDown : [status8 == true && Sensors_70.O_70_Pist_Back == true]
    Identified_Delivery.InitialCondition -> Identified_Delivery.Part_Arrives : [status == true && Sensors_70.O_70_SPart == true]
    Identified_Delivery.Elevator_MiddleDown -> Identified_Delivery.Elevator_InductiveDown : [status11 == true && Sensors_70.O_70_SInductive == true]
    Identified_Delivery.Part_Arrives -> Identified_Delivery.Elevator_Up : [status1 == true && Sensors_80.O_80_Arm_Mag == true ]
    Identified_Delivery.Elevator_High -> Identified_Delivery.Part_HeightSensor [order 2] : [status5 == true && status6 == true && Sensors_70.O_70_Pist_Back == false]
    Identified_Delivery.Elevator_InductiveDown -> Identified_Delivery.Elevator_Down : [status12 == true && Sensors_70.O_70_Elev_Low == true]
    Identified_Delivery.Elevator_Down -> Identified_Delivery.End_Process : after (2,sec)
    Identified_Delivery.Part_HeightSensor -> Identified_Delivery.Part_ArrivesAtCart [order 2] : [status7 == true && AS_i_70.A_74_Optic == true]
    Identified_Delivery.Elevator_High -> Identified_Delivery.Pushes_Part [order 1] : after (2,sec)
  state Distribution_Continuous
    state InitialCondition
      entry:
      status = false;
      during:
      Sensors_70.O_70_SStation
      Control_70.C_75_RQ_Wrong
      AS_i_70.A_74_CRoute_In80
      Control_80.C_85_Single
      Control_80.C_85_Start
      Control_80.C_85_Part_Del
      Control_80.C_86_Mag_Parts
      Actuators_80.F_82_Pist_Adv
      Actuators_80.F_82_Arm_2_Del
      Actuators_80.F_82_Arm_2_Mag
      Actuators_80.F_82_Suction_On
      Actuators_80.F_82_Suction_Off
      Actuators_80.F_83_Led_Extra1
      Sensors_80.O_80_Arm_Mag
      Sensors_80.O_80_Arm_Del
      Sensors_80.O_80_Pist_Back
      Sensors_80.O_80_Pist_Fwd
      Sensors_80.O_80_Part_Stuck
      Sensors_80.O_81_Start
      Sensors_80.O_81_Key_Pos
      if ~Sensors_70.O_70_SStation && ...
      ~Control_70.C_75_RQ_Wrong && ...
      ~AS_i_70.A_74_CRoute_In80 && ...
      Control_80.C_85_Single && ...
      ~Control_80.C_85_Start && ...
      ~Control_80.C_85_Part_Del && ...
      Control_80.C_86_Mag_Parts ~= 0 && ...
      ~Actuators_80.F_82_Pist_Adv && ...
      ~Actuators_80.F_82_Arm_2_Del && ...
      ~Actuators_80.F_82_Arm_2_Mag && ...
      ~Actuators_80.F_82_Suction_On && ...
      ~Actuators_80.F_82_Suction_Off && ...
      ~Actuators_80.F_83_Led_Extra1 && ...
      Sensors_80.O_80_Arm_Mag && ...
      ~Sensors_80.O_80_Arm_Del && ...
      Sensors_80.O_80_Pist_Back && ...
      ~Sensors_80.O_80_Pist_Fwd && ...
      ~Sensors_80.O_80_Part_Stuck && ...
      ~Sensors_80.O_81_Start && ...
      Sensors_80.O_81_Key_Pos
      status = true;
      else
      status = false;
      end
    state ArmToDelivery
      entry:
      status1 = false;
      during:
      Actuators_80.F_82_Arm_2_Del
      if Actuators_80.F_82_Arm_2_Del
      status1 = true;
      else
      status1 = false;
      end
    state ArmArrives_FeedsPart
      entry:
      status3 = false;
      during:
      Actuators_80.F_82_Pist_Adv
      Actuators_80.F_82_Arm_2_Del
      Sensors_80.O_80_Arm_Del
      if Actuators_80.F_82_Pist_Adv && ...
      ~Actuators_80.F_82_Arm_2_Del && ...
      Sensors_80.O_80_Arm_Del
      status3 = true;
      else
      status3 = false;
      end
    state PartFed
      entry:
      status5 = false;
      during:
      Control_80.C_86_Mag_Parts
      Actuators_80.F_82_Pist_Adv
      Sensors_80.O_80_Pist_Fwd
      if Control_80.C_86_Mag_Parts ~= 0 && ...
      ~Actuators_80.F_82_Pist_Adv && ...
      Sensors_80.O_80_Pist_Fwd
      status5 = true;
      else
      status5 = false;
      end
    state ArmToMagazine
      entry:
      status7 = false;
      during:
      Actuators_80.F_82_Arm_2_Mag
      if Actuators_80.F_82_Arm_2_Mag
      status7 = true;
      else
      status7 = false;
      end
    state ArmArrives_PicksPart
      entry:
      status9 = false;
      during:
      Actuators_80.F_82_Arm_2_Mag
      Actuators_80.F_82_Suction_On
      if ~Actuators_80.F_82_Arm_2_Mag && ...
      Actuators_80.F_82_Suction_On
      status9 = true;
      else
      status9 = false;
      end
    state ArmToDelivery1
      entry:
      status10 = false;
      during:
      Actuators_80.F_82_Arm_2_Del
      if Actuators_80.F_82_Arm_2_Del
      status10 = true;
      else
      status10 = false;
      end
    state ArmArrives_DeliversPart
      entry:
      status12 = false;
      during:
      Actuators_80.F_82_Arm_2_Del
      Actuators_80.F_82_Suction_On
      Actuators_80.F_82_Suction_Off
      if ~Actuators_80.F_82_Arm_2_Del && ...
      ~Actuators_80.F_82_Suction_On && ...
      Actuators_80.F_82_Suction_Off
      status12 = true;
      else
      status12 = false;
      end
    state PartDel_CheckLoop
      entry:
      LoopDistCont = false;
      during:
      Control_80.C_85_Part_Del
      Actuators_80.F_82_Arm_2_Mag
      Actuators_80.F_82_Suction_Off
      Actuators_80.F_83_Led_Extra1
      Control_80.C_86_Mag_Parts
      if Control_80.C_85_Part_Del && ...
      Actuators_80.F_83_Led_Extra1 && ...
      Control_80.C_86_Mag_Parts ~= 0
      LoopDistCont = true;
      else
      LoopDistCont = false;
      end
    state ArmToMagazine1
      entry:
      status13 = false;
      during:
      Actuators_80.F_82_Arm_2_Mag
      if Actuators_80.F_82_Arm_2_Mag
      status13 = true;
      else
      status13 = false;
      end
    state ArmArrives_Finish
      during:
      Actuators_80.F_82_Arm_2_Mag
    state ArmCloseDelivery
      entry:
      status2 = false;
      during:
      Sensors_70.O_70_SStation
      if Sensors_70.O_70_SStation
      status2 = true;
      else
      status2 = false;
      end
    state PistonStartsMoveForward
      entry:
      status4 = false;
      during:
      Sensors_80.O_80_Pist_Back
      if ~Sensors_80.O_80_Pist_Back
      status4 = true;
      else
      status4 = false;
      end
    state PistonStartsMoveBackward
      entry:
      status6 = false;
      during:
      Sensors_80.O_80_Pist_Fwd
      if ~Sensors_80.O_80_Pist_Fwd
      status6 = true;
      else
      status6 = false;
      end
    state ArmCloseDeliver1
      entry:
      status8 = false;
      during:
      Sensors_70.O_70_SStation
      if ~Sensors_70.O_70_SStation
      status8 = true;
      else
      status8 = false;
      end
    state ArmCloseDelivery3
      entry:
      status11 = false;
      during:
      Sensors_70.O_70_SStation
      if Sensors_70.O_70_SStation
      status11 = true;
      else
      status11 = false;
      end
    state ArmCloseDeliver4
      entry:
      status14 = false;
      during:
      Sensors_70.O_70_SStation
      if ~Sensors_70.O_70_SStation
      status14 = true;
      else
      status14 = false;
      end
    state T1
      during:
      Control_80.C_85_Part_Del
      Actuators_80.F_83_Led_Extra1
    (default) -> Distribution_Continuous.InitialCondition
    Distribution_Continuous.ArmToDelivery1 -> Distribution_Continuous.ArmArrives_DeliversPart [order 2] : [Sensors_80.O_80_Arm_Del == true && ...
        | status11 == true]
    Distribution_Continuous.ArmArrives_DeliversPart -> Distribution_Continuous.PartDel_CheckLoop : [Sensors_80.O_80_Part_Stuck == false && ...
        | status12 == true]
    Distribution_Continuous.ArmToMagazine -> Distribution_Continuous.ArmArrives_PicksPart [order 2] : [Sensors_80.O_80_Arm_Mag == true && ...
        | status8 == true]
    Distribution_Continuous.ArmArrives_PicksPart -> Distribution_Continuous.ArmToDelivery1 : [Sensors_80.O_80_Part_Stuck == true && ...
        | status9 == true]
    Distribution_Continuous.PartDel_CheckLoop -> Distribution_Continuous.ArmToMagazine1 [order 2] : [LoopDistCont == false]
    Distribution_Continuous.ArmToDelivery -> Distribution_Continuous.ArmArrives_FeedsPart [order 2] : [Sensors_80.O_80_Arm_Del == true && ...
        | status2 == true]
    Distribution_Continuous.ArmToMagazine1 -> Distribution_Continuous.ArmArrives_Finish [order 1] : [Sensors_80.O_80_Arm_Mag == true && ...
        | status14 == true]
    Distribution_Continuous.ArmArrives_FeedsPart -> Distribution_Continuous.PartFed [order 2] : [Sensors_80.O_80_Pist_Fwd == true && ...
        | status4 == true]
    Distribution_Continuous.PartFed -> Distribution_Continuous.ArmToMagazine [order 2] : [Sensors_80.O_80_Pist_Back == true && ...
        | status6 == true]
    Distribution_Continuous.InitialCondition -> Distribution_Continuous.ArmToDelivery : [Sensors_80.O_81_Start == true | ...
        | Control_80.C_85_Start == true | ...
        | Control_70.C_75_RQ_Wrong == true | ...
        | (AS_i_70.A_74_CRoute_In80 == true && Sensors_80.O_81_Key_Pos == true) ]
    (junction 708) -> Distribution_Continuous.ArmArrives_FeedsPart
    Distribution_Continuous.ArmToDelivery -> Distribution_Continuous.ArmCloseDelivery [order 1] : [Sensors_80.O_80_Arm_Mag == false &&...
        |  status1 == true]
    (junction 706) -> (junction 708)
    Distribution_Continuous.ArmToDelivery1 -> ArmCloseDelivery3 [order 1] : [Sensors_80.O_80_Arm_Mag == false &&...
        |  status10 == true]
    Distribution_Continuous.ArmToMagazine -> Distribution_Continuous.ArmCloseDeliver1 [order 1] : [Sensors_80.O_80_Arm_Del == false &&...
        |  status7 == true]
    Distribution_Continuous.ArmArrives_FeedsPart -> Distribution_Continuous.PistonStartsMoveForward [order 1] : [status3 == true]
    Distribution_Continuous.PartFed -> Distribution_Continuous.PistonStartsMoveBackward [order 1] : [status5 == true]
    Distribution_Continuous.ArmToMagazine1 -> Distribution_Continuous.ArmCloseDeliver4 [order 2] : [Sensors_80.O_80_Arm_Del == false &&...
        |  status13 == true]
    Distribution_Continuous.PartDel_CheckLoop -> (junction 707) [order 1] : [LoopDistCont == true]
    Distribution_Continuous.PartDel_CheckLoop -> Distribution_Continuous.T1 [order 3] : after(4,sec)
    (junction 707) -> (junction 706)
  state Requested_Delivery
    state Part_HeightSensor
      entry:
      status7 = false;
      during:
      Actuators_70.F_72_Eject_Part;
      Sensors_70.O_70_Pist_Back;
      Sensors_70.O_70_SPart_Height
      if Actuators_70.F_72_Eject_Part && ...
      ~Sensors_70.O_70_Pist_Back && ...
      ~Sensors_70.O_70_SPart_Height
      status7 = true
      else
      status7 = false
      end
    state Piston_Back
      entry:
      status8 = false;
      during:
      Actuators_70.F_72_Eject_Part
      if ~Actuators_70.F_72_Eject_Part
      status8 = true
      else
      status8 = false
      end
    state Elevator_StartsMovingDown
      entry:
      status10 = false;
      during:
      Actuators_70.F_72_Elev_Down;
      Actuators_70.F_72_Elev_Up;
      if Actuators_70.F_72_Elev_Down && ...
      ~Actuators_70.F_72_Elev_Up
      status10 = true
      else
      status10 = false
      end
    state Elevator_MiddleDown
      entry:
      status11 = false;
      during:
      Sensors_70.O_70_SStation;
      if ~Sensors_70.O_70_SStation
      status11 = true
      else
      status11 = false
      end
    state Elevator_InductiveDown
      entry:
      status12 = false;
      during:
      Sensors_70.O_70_SInductive;
      if ~Sensors_70.O_70_SInductive
      status12 = true
      else
      status12 = false
      end
    state Elevator_Down
      entry:
      status13 = false;
      during:
      AS_i_70.A_74_CRoute_Out;
      Actuators_70.F_72_Elev_Down;
      Control_70.C_75_Part_Del;
      if AS_i_70.A_74_CRoute_Out && ...
      ~Actuators_70.F_72_Elev_Down&& ...
      Control_70.C_75_Part_Del
      status13 = true
      else
      status13 = false
      end
    state InitialCondition
      entry:
      status = false;
      during:
      AS_i_70.A_74_Cart_Full;
      AS_i_70.A_74_CRoute_Out;
      AS_i_70.A_74_Optic;
      Control_70.C_75_ID_Delivery1;
      Control_70.C_75_ID_Delivery2;
      Control_70.C_75_Requested;
      Control_70.C_75_RQ_Part_Del;
      Control_70.C_75_RQ_Wrong;
      Control_70.C_75_RQ_Delivery1;
      Control_70.C_75_RQ_Delivery2;
      Actuators_70.F_72_Elev_Down;
      Actuators_70.F_72_Elev_Up;
      Actuators_70.F_72_Eject_Part;
      Actuators_70.F_72_Air_On;
      Actuators_70.F_73_Led_Extra1;
      Actuators_70.F_73_Led_Extra2;
      Sensors_70.O_70_SInductive;
      Sensors_70.O_70_SPart;
      Sensors_70.O_70_SStation;
      Sensors_70.O_70_SPart_Height;
      Sensors_70.O_70_Elev_High;
      Sensors_70.O_70_Elev_Low;
      Sensors_70.O_70_Pist_Back;
      Sensors_70.O_71_Start;
      Sensors_70.O_71_Stop;
      Sensors_70.O_71_Key_Pos;
      Sensors_70.O_71_Reset;
      Sensors_80.O_80_Arm_Mag
      if Control_70.C_75_Requested && ...
      ~Sensors_70.O_70_SPart && ...
      ~Sensors_80.O_80_Arm_Mag
      status = true;
      else
      status = false;
      end
    state Part_Arrives
      entry:
      status1 == false;
      MetalicPart == false;
      during:
      Control_70.C_75_ID_Delivery2;
      Sensors_70.O_70_SInductive;
      Sensors_70.O_70_SPart;
      Sensors_80.O_80_Arm_Mag
      if Sensors_70.O_70_SInductive
      MetalicPart = true
      else
      MetalicPart = false
      end
      if Sensors_70.O_70_SPart && ...
      ((Sensors_70.O_70_SInductive && ...
      Control_70.C_75_ID_Delivery2) | ...
      (~Sensors_70.O_70_SInductive && ...
      ~Control_70.C_75_ID_Delivery2)) && ...
      ~Sensors_80.O_80_Arm_Mag
      status1 = true;
      else
      status1 =false;
      end
    state Elevator_Up
      entry:
      status2 = false
      during:
      Actuators_70.F_72_Elev_Up;
      if Actuators_70.F_72_Elev_Up
      status2 = true
      else
      status2 = false
      end
    state Elevator_StartsMovingUp
      entry:
      status3 = false;
      during:
      Sensors_70.O_70_SInductive;
      if ~Sensors_70.O_70_SInductive
      status3 = true
      else
      status3 = false
      end
    state Elevator_MiddleUp
      entry:
      status4 = false;
      during:
      Sensors_70.O_70_SStation;
      if ~Sensors_70.O_70_SStation
      status4 = true
      else
      status4 = false
      end
    state Elevator_High
      entry:
      status5 = false;
      during:
      MetalicPart;
      Control_70.C_75_ID_Delivery1;
      Control_70.C_75_ID_Delivery2;
      Sensors_70.O_70_SPart_Height;
      if MetalicPart && ...
      Control_70.C_75_ID_Delivery2 && ...
      ~Control_70.C_75_ID_Delivery1;
      status5 = true
      end
      if ~MetalicPart && ...
      Control_70.C_75_ID_Delivery1 && ...
      ((Sensors_70.O_70_SPart_Height && ...
      Control_70.C_75_ID_Delivery2) | ...
      (~Sensors_70.O_70_SPart_Height && ...
      ~Control_70.C_75_ID_Delivery2))
      status5=true
      end
    state CheckPart
      entry:
      Part_Equal = false;
      Part_Different = false;
      during:
      Control_70.C_75_ID_Delivery1;
      Control_70.C_75_ID_Delivery2;
      Control_70.C_75_RQ_Delivery1;
      Control_70.C_75_RQ_Delivery2;
      if (Control_70.C_75_ID_Delivery1 == ...
      Control_70.C_75_RQ_Delivery1) && ...
      (Control_70.C_75_ID_Delivery2 == ...
      Control_70.C_75_RQ_Delivery2)
      Part_Equal = true
      else
      Part_Different = true
      end
    state Pushes_Part
      entry:
      status6 = false;
      during:
      Actuators_70.F_72_Eject_Part;
      Actuators_70.F_72_Air_On;
      Sensors_70.O_70_SPart
      if Actuators_70.F_72_Eject_Part && ...
      Actuators_70.F_72_Air_On && ...
      ~Sensors_70.O_70_SStation
      status6 = true
      else
      status6 = false
      end
    state Part_ArrivesAtCart
      entry:
      status9 = false;
      during:
      AS_i_70.A_74_Cart_Full;
      AS_i_70.A_74_Optic;
      Actuators_70.F_72_Air_On;
      Actuators_70.F_73_Led_Extra2
      if AS_i_70.A_74_Optic && ...
      AS_i_70.A_74_Cart_Full && ...
      ~Actuators_70.F_72_Air_On && ...
      Actuators_70.F_73_Led_Extra2;
      status9 = true
      else
      status9 = false
      end
    state End_Process
      entry:
      status14 = false;
      during:
      AS_i_70.A_74_CRoute_Out;
      if  ~AS_i_70.A_74_CRoute_Out;
      status14 = true
      else
      status14 = false
      end
    state Elevator_StartsMovingDown1
      entry:
      status15 = false;
      during:
      Actuators_70.F_72_Elev_Down;
      Actuators_70.F_72_Elev_Up;
      if Actuators_70.F_72_Elev_Down && ...
      ~Actuators_70.F_72_Elev_Up
      status15 = true
      else
      status15 = false
      end
    state Elevator_MiddleDown1
      entry:
      status16 = false;
      during:
      Sensors_70.O_70_SStation;
      if ~Sensors_70.O_70_SStation
      status16 = true
      else
      status16 = false
      end
    state Elevator_InductiveDown1
      entry:
      status17 = false;
      during:
      Sensors_70.O_70_SInductive;
      if ~Sensors_70.O_70_SInductive
      status17 = true
      else
      status17 = false
      end
    state Elevator_Down1
      entry:
      status18 = false;
      during:
      Actuators_70.F_72_Eject_Part
      Actuators_70.F_72_Elev_Down
      if Actuators_70.F_72_Eject_Part && ...
      ~Actuators_70.F_72_Elev_Down
      status18 = true
      else
      status18 = false
      end
    state Piston_Back1
      entry:
      status19 = false;
      during:
      Actuators_70.F_72_Eject_Part
      Sensors_70.O_70_Pist_Back;
      Sensors_70.O_70_SPart
      Control_70.C_75_RQ_Wrong;
      if ~Actuators_70.F_72_Eject_Part && ...
      Sensors_70.O_70_Pist_Back && ...
      ~Sensors_70.O_70_SPart && ...
      Control_70.C_75_RQ_Wrong;
      status19 = true
      else
      status19 = false
      end
    (default) -> Requested_Delivery.InitialCondition
    Requested_Delivery.Part_HeightSensor -> Requested_Delivery.Piston_Back [order 2] : after (2,sec)
    Requested_Delivery.Elevator_StartsMovingDown -> Requested_Delivery.Elevator_MiddleDown : [status10 == true && Sensors_70.O_70_SStation == true]
    Requested_Delivery.Pushes_Part -> Requested_Delivery.Part_HeightSensor : [status6 == true && Sensors_70.O_70_SPart_Height == true]
    Requested_Delivery.Piston_Back -> Requested_Delivery.Elevator_StartsMovingDown : [status8 == true && Sensors_70.O_70_Pist_Back == true]
    Requested_Delivery.Elevator_High -> CheckPart : [status5 == true]
    Requested_Delivery.Elevator_StartsMovingUp -> Requested_Delivery.Elevator_MiddleUp : [status3 == true && Sensors_70.O_70_SStation == true]
    Requested_Delivery.Elevator_MiddleUp -> Requested_Delivery.Elevator_High : [status4 == true && Sensors_70.O_70_Elev_High == true]
    Requested_Delivery.Elevator_Up -> Requested_Delivery.Elevator_StartsMovingUp : [status2 == true && Sensors_70.O_70_SInductive == true ]
    Requested_Delivery.Elevator_MiddleDown -> Requested_Delivery.Elevator_InductiveDown : [status11 == true && Sensors_70.O_70_SInductive == true]
    Requested_Delivery.InitialCondition -> Requested_Delivery.Part_Arrives : [status == true && Sensors_70.O_70_SPart == true]
    CheckPart -> Requested_Delivery.Pushes_Part [order 1] : [Part_Equal == true && after (2,sec)]
    Requested_Delivery.Part_Arrives -> Requested_Delivery.Elevator_Up : [status1 == true && Sensors_80.O_80_Arm_Mag == true ]
    Requested_Delivery.Elevator_InductiveDown -> Requested_Delivery.Elevator_Down : [status12 == true && Sensors_70.O_70_Elev_Low == true]
    Requested_Delivery.Elevator_Down -> Requested_Delivery.End_Process : after (2,sec)
    Requested_Delivery.Part_HeightSensor -> Requested_Delivery.Part_ArrivesAtCart [order 1] : [status7 == true && AS_i_70.A_74_Optic == true]
    CheckPart -> (junction 952) [order 2] : [Part_Different == true && after (2,sec)]
    Elevator_MiddleDown1 -> Elevator_InductiveDown1 : [status16 == true && Sensors_70.O_70_SInductive == true]
    Elevator_StartsMovingDown1 -> Elevator_MiddleDown1 : [status15 == true && Sensors_70.O_70_SStation == true]
    Elevator_Down1 -> Piston_Back1 : [status18 == true && Sensors_70.O_70_Pist_Back == false]
    Elevator_InductiveDown1 -> Elevator_Down1 : [status12 == true && Sensors_70.O_70_Elev_Low == true]
    (junction 952) -> Elevator_StartsMovingDown1
  state Distribution_Counted
    state InitialCondition
      entry:
      status = false;
      during:
      AS_i_70.A_74_CRoute_In80
      Control_70.C_75_RQ_Part_Del
      Control_70.C_75_Identified80
      Control_70.C_75_Requested80
      Sensors_70.O_70_SStation
      Actuators_80.F_82_Pist_Adv
      Actuators_80.F_82_Arm_2_Del
      Actuators_80.F_82_Arm_2_Mag
      Actuators_80.F_82_Suction_On
      Actuators_80.F_82_Suction_Off
      Actuators_80.F_83_Led_Extra1
      Control_80.C_85_Counted
      Control_80.C_85_Start
      Control_80.C_85_Part_Del
      Control_80.C_86_Mag_Parts
      Control_80.C_83_RQ_Parts
      Control_80.C_87_RQ_MParts
      Sensors_80.O_80_Arm_Mag
      Sensors_80.O_80_Arm_Del
      Sensors_80.O_80_Pist_Back
      Sensors_80.O_80_Pist_Fwd
      Sensors_80.O_80_Part_Stuck
      Sensors_80.O_81_Start
      Sensors_80.O_81_Key_Pos
      if ~AS_i_70.A_74_CRoute_In80 && ...
      ~Sensors_70.O_70_SStation && ...
      ~Actuators_80.F_82_Pist_Adv && ...
      ~Actuators_80.F_82_Arm_2_Del && ...
      ~Actuators_80.F_82_Arm_2_Mag && ...
      ~Actuators_80.F_82_Suction_On && ...
      ~Actuators_80.F_82_Suction_Off && ...
      ~Actuators_80.F_83_Led_Extra1 && ...
      Control_80.C_83_RQ_Parts ~= 0 && ...
      Control_80.C_85_Counted && ...
      ~Control_80.C_85_Start && ...
      ~Control_80.C_85_Part_Del && ...
      Control_80.C_86_Mag_Parts ~= 0 && ...
      Control_80.C_87_RQ_MParts ~= 0 && ...
      Sensors_80.O_80_Arm_Mag && ...
      ~Sensors_80.O_80_Arm_Del && ...
      Sensors_80.O_80_Pist_Back && ...
      ~Sensors_80.O_80_Pist_Fwd && ...
      ~Sensors_80.O_80_Part_Stuck && ...
      ~Sensors_80.O_81_Start && ...
      Sensors_80.O_81_Key_Pos
      status = true;
      else
      status = false;
      end
    state ArmToDelivery
      entry:
      status1 = false;
      during:
      Actuators_80.F_82_Arm_2_Del
      if Actuators_80.F_82_Arm_2_Del
      status1 = true;
      else
      status1 = false;
      end
    state ArmArrives_FeedsPart
      entry:
      status3 = false;
      during:
      Actuators_80.F_82_Pist_Adv
      Actuators_80.F_82_Arm_2_Del
      Sensors_80.O_80_Arm_Del
      if Actuators_80.F_82_Pist_Adv && ...
      ~Actuators_80.F_82_Arm_2_Del && ...
      Sensors_80.O_80_Arm_Del
      status3 = true;
      else
      status3 = false;
      end
    state PartFed
      entry:
      status5 = false;
      during:
      Control_80.C_86_Mag_Parts
      Actuators_80.F_82_Pist_Adv
      Sensors_80.O_80_Pist_Fwd
      if Control_80.C_86_Mag_Parts ~= 0 && ...
      ~Actuators_80.F_82_Pist_Adv && ...
      Sensors_80.O_80_Pist_Fwd
      status5 = true;
      else
      status5 = false;
      end
    state ArmToMagazine
      entry:
      status7 = false;
      during:
      Actuators_80.F_82_Arm_2_Mag
      if Actuators_80.F_82_Arm_2_Mag
      status7 = true;
      else
      status7 = false;
      end
    state ArmArrives_PicksPart
      entry:
      status9 = false;
      during:
      Actuators_80.F_82_Arm_2_Mag
      Actuators_80.F_82_Suction_On
      if ~Actuators_80.F_82_Arm_2_Mag && ...
      Actuators_80.F_82_Suction_On
      status9 = true;
      else
      status9 = false;
      end
    state ArmToDelivery1
      entry:
      status10 = false;
      during:
      Actuators_80.F_82_Arm_2_Del
      if Actuators_80.F_82_Arm_2_Del
      status10 = true;
      else
      status10 = false;
      end
    state ArmArrives_DeliversPart1
      entry:
      status12 = false;
      during:
      Actuators_80.F_82_Arm_2_Del
      Actuators_80.F_82_Suction_On
      Actuators_80.F_82_Suction_Off
      if ~Actuators_80.F_82_Arm_2_Del && ...
      ~Actuators_80.F_82_Suction_On && ...
      Actuators_80.F_82_Suction_Off
      status12 = true;
      else
      status12 = false;
      end
    state PartDel_CheckLoop
      entry:
      LoopDistCont = false;
      during:
      Control_80.C_85_Part_Del
      Actuators_80.F_82_Arm_2_Mag
      Actuators_80.F_82_Suction_Off
      Actuators_80.F_83_Led_Extra1
      Control_80.C_87_RQ_MParts
      if Control_80.C_85_Part_Del && ...
      Control_80.C_87_RQ_MParts == 0
      LoopDistCont = true;
      else
      LoopDistCont = false;
      end
    state ArmToMagazine1
      entry:
      status13 = false;
      during:
      Actuators_80.F_82_Arm_2_Mag
      if Actuators_80.F_82_Arm_2_Mag
      status13 = true;
      else
      status13 = false;
      end
    state ArmArrives_Finish
      during:
      Actuators_80.F_82_Arm_2_Mag
    state ArmCloseDelivery
      entry:
      status2 = false;
      during:
      Sensors_70.O_70_SStation
      if Sensors_70.O_70_SStation
      status2 = true;
      else
      status2 = false;
      end
    state PistonStartsMoveForward
      entry:
      status4 = false;
      during:
      Sensors_80.O_80_Pist_Back
      if ~Sensors_80.O_80_Pist_Back
      status4 = true;
      else
      status4 = false;
      end
    state PistonStartsMoveBackward
      entry:
      status6 = false;
      during:
      Sensors_80.O_80_Pist_Fwd
      if ~Sensors_80.O_80_Pist_Fwd
      status6 = true;
      else
      status6 = false;
      end
    state ArmCloseDeliver1
      entry:
      status8 = false;
      during:
      Sensors_70.O_70_SStation
      if ~Sensors_70.O_70_SStation
      status8 = true;
      else
      status8 = false;
      end
    state ArmCloseDelivery2
      entry:
      status11 = false;
      during:
      Sensors_70.O_70_SStation
      if Sensors_70.O_70_SStation
      status11 = true;
      else
      status11 = false;
      end
    state ArmCloseDeliver4
      entry:
      status14 = false;
      during:
      Sensors_70.O_70_SStation
      if ~Sensors_70.O_70_SStation
      status14 = true;
      else
      status14 = false;
      end
    state T2
      during:
      Control_80.C_85_Part_Del
      Actuators_80.F_83_Led_Extra1
    (default) -> Distribution_Counted.InitialCondition
    Distribution_Counted.ArmToDelivery1 -> ArmArrives_DeliversPart1 [order 2] : [Sensors_80.O_80_Arm_Del == true && ...
        | status11 == true]
    Distribution_Counted.InitialCondition -> Distribution_Counted.ArmToDelivery : [Sensors_80.O_81_Start == true | ...
        | Control_80.C_85_Start == true | ...
        | Control_70.C_75_RQ_Wrong == true | ...
        | (AS_i_70.A_74_CRoute_In80 == true && Sensors_80.O_81_Key_Pos == true) ]
    ArmArrives_DeliversPart1 -> Distribution_Counted.PartDel_CheckLoop : [Sensors_80.O_80_Part_Stuck == false && ...
        | status12 == true]
    Distribution_Counted.ArmToMagazine -> Distribution_Counted.ArmArrives_PicksPart [order 2] : [Sensors_80.O_80_Arm_Mag == true && ...
        | status8 == true]
    Distribution_Counted.ArmArrives_PicksPart -> Distribution_Counted.ArmToDelivery1 : [Sensors_80.O_80_Part_Stuck == true && ...
        | status9 == true]
    Distribution_Counted.PartDel_CheckLoop -> Distribution_Counted.ArmToMagazine1 [order 2] : [LoopDistCont == false]
    Distribution_Counted.ArmToDelivery -> Distribution_Counted.ArmArrives_FeedsPart [order 2] : [Sensors_80.O_80_Arm_Del == true && ...
        | status2 == true]
    Distribution_Counted.ArmToMagazine1 -> Distribution_Counted.ArmArrives_Finish [order 1] : [Sensors_80.O_80_Arm_Mag == true && ...
        | status14 == true]
    Distribution_Counted.ArmArrives_FeedsPart -> Distribution_Counted.PartFed [order 2] : [Sensors_80.O_80_Pist_Fwd == true && ...
        | status4 == true]
    Distribution_Counted.PartFed -> Distribution_Counted.ArmToMagazine [order 2] : [Sensors_80.O_80_Pist_Back == true && ...
        | status6 == true]
    (junction 804) -> Distribution_Counted.ArmArrives_FeedsPart
    Distribution_Counted.ArmToDelivery -> Distribution_Counted.ArmCloseDelivery [order 1] : [Sensors_80.O_80_Arm_Mag == false &&...
        |  status1 == true]
    (junction 820) -> (junction 804)
    Distribution_Counted.ArmToDelivery1 -> Distribution_Counted.ArmCloseDelivery2 [order 1] : [Sensors_80.O_80_Arm_Mag == false &&...
        |  status10 == true]
    Distribution_Counted.ArmToMagazine -> Distribution_Counted.ArmCloseDeliver1 [order 1] : [Sensors_80.O_80_Arm_Del == false &&...
        |  status7 == true]
    Distribution_Counted.ArmArrives_FeedsPart -> Distribution_Counted.PistonStartsMoveForward [order 1] : [status3 == true]
    Distribution_Counted.PartFed -> Distribution_Counted.PistonStartsMoveBackward [order 1] : [status5 == true]
    Distribution_Counted.ArmToMagazine1 -> Distribution_Counted.ArmCloseDeliver4 [order 2] : [Sensors_80.O_80_Arm_Del == false &&...
        |  status13 == true]
    Distribution_Counted.PartDel_CheckLoop -> (junction 821) [order 1] : [LoopDistCont == true]
    Distribution_Counted.PartDel_CheckLoop -> Distribution_Counted.T2 [order 3] : after(4,sec)
    (junction 821) -> (junction 820)
  state CartToProcessing
    state InitialCondition
      entry:
      status = false;
      during:
      Control_20.C_25_Request
      Actuators_20.F_22_Conveyor
      Actuators_20.F_24_Release_FB
      AS_i_70.A_74_Release_FB
      AS_i_70.A_73_SortCartID
      Sensors_20.O_24_Pist_Back
      AS_i_70.A_74_Pist_Bck
      Sensors_20.O_24_Cart_Stat
      AS_i_70.A_74_Cart_Stat
      AS_i_70.A_74_No_Cart
      Actuators_70.F_73_Led_Extra1
      Sensors_20.O_24_Cart_Next
      AS_i_70.A_74_Cart_Next
      AS_i_90.A_93_TestCartID
      Sensors_20.O_25_Cart_Stat
      AS_i_90.A_94_Cart_Stat
      Control_20.C_25_CartDel
      AS_i_90.A_94_No_Cart
      Actuators_90.F_93_Led_Extra1
      AS_i_90.A_94_CRoute_In
      if ~Control_20.C_25_Request && ...
      ~Actuators_20.F_22_Conveyor && ...
      ~Actuators_20.F_24_Release_FB && ...
      ~AS_i_70.A_74_Release_FB && ...
      AS_i_70.A_73_SortCartID ~= 0 && ...
      ~Sensors_20.O_24_Pist_Back && ...
      ~AS_i_70.A_74_Pist_Bck && ...
      Sensors_20.O_24_Cart_Stat && ...
      AS_i_70.A_74_Cart_Stat && ...
      ~AS_i_70.A_74_No_Cart && ...
      ~Actuators_70.F_73_Led_Extra1 && ...
      ~Sensors_20.O_24_Cart_Next && ...
      ~AS_i_70.A_74_Cart_Next && ...
      AS_i_90.A_93_TestCartID == 0 && ...
      ~Sensors_20.O_25_Cart_Stat && ...
      ~AS_i_90.A_94_Cart_Stat && ...
      ~Control_20.C_25_CartDel && ...
      AS_i_90.A_94_No_Cart && ...
      Actuators_90.F_93_Led_Extra1 && ...
      ~AS_i_90.A_94_CRoute_In
      status = true;
      else
      status = false;
      end
    state StartsProcess
      entry:
      status2 = false;
      during:
      Control_20.C_25_Request;
      Actuators_20.F_22_Conveyor;
      Actuators_20.F_24_Release_FB;
      AS_i_70.A_74_Release_FB;
      AS_i_70.A_73_SortCartID;
      Sensors_20.O_24_Pist_Back;
      AS_i_70.A_74_Pist_Bck;
      if Control_20.C_25_Request && ...
      Actuators_20.F_22_Conveyor && ...
      Actuators_20.F_24_Release_FB && ...
      AS_i_70.A_74_Release_FB && ...
      AS_i_70.A_73_SortCartID == 0 && ...
      Sensors_20.O_24_Pist_Back && ...
      AS_i_70.A_74_Pist_Bck
      status2 = true;
      else
      status2 = false;
      end
    state CartStartsMoving
      entry:
      status3 = false;
      during:
      Sensors_20.O_24_Cart_Stat
      AS_i_70.A_74_Cart_Stat
      AS_i_70.A_74_No_Cart
      Actuators_70.F_73_Led_Extra1
      if ~Sensors_20.O_24_Cart_Stat && ...
      ~AS_i_70.A_74_Cart_Stat && ...
      AS_i_70.A_74_No_Cart && ...
      Actuators_70.F_73_Led_Extra1
      status3 = true;
      else
      status3 = false;
      end
    state CartGetsNearNextStation
      entry:
      status4 = false;
      during:
      Actuators_20.F_24_Release_FB
      AS_i_70.A_74_Release_FB
      Sensors_20.O_24_Pist_Back
      AS_i_70.A_74_Pist_Bck
      Sensors_20.O_24_Cart_Next
      AS_i_70.A_74_Cart_Next
      if ~Actuators_20.F_24_Release_FB && ...
      ~AS_i_70.A_74_Release_FB && ...
      ~Sensors_20.O_24_Pist_Back && ...
      ~AS_i_70.A_74_Pist_Bck && ...
      Sensors_20.O_24_Cart_Next && ...
      AS_i_70.A_74_Cart_Next
      status4 = true;
      else
      status4 = false;
      end
    state DetectionofCartNumberinStation
      entry:
      status5 = false;
      during:
      AS_i_90.A_93_TestCartID
      if ~AS_i_90.A_93_TestCartID
      status5 = true;
      end
    state CartPassesNextStation
      entry:
      status6 = false;
      during:
      Sensors_20.O_24_Cart_Next
      AS_i_70.A_74_Cart_Next
      if ~Sensors_20.O_24_Cart_Next && ...
      ~AS_i_70.A_74_Cart_Next
      status6 = true;
      else
      status6 = false;
      end
    state CartArrivesinNextStation
      entry:
      status7 = false;
      during:
      Sensors_20.O_25_Cart_Stat
      AS_i_90.A_94_Cart_Stat
      Control_20.C_25_CartDel
      AS_i_90.A_94_No_Cart
      Actuators_90.F_93_Led_Extra1
      AS_i_90.A_94_CRoute_In
      if Sensors_20.O_25_Cart_Stat &&...
      AS_i_90.A_94_Cart_Stat &&...
      Control_20.C_25_CartDel &&...
      ~AS_i_90.A_94_No_Cart &&...
      ~Actuators_90.F_93_Led_Extra1 &&...
      AS_i_90.A_94_CRoute_In
      status7 = true;
      else
      status7 = false;
      end
    state T3
      during:
      Control_20.C_25_CartDel
    state T2
      during:
      AS_i_90.A_94_CRoute_In
    state T1
      during:
      Control_20.C_25_Request
    (default) -> CartToProcessing.InitialCondition
    CartToProcessing.CartStartsMoving -> CartToProcessing.CartGetsNearNextStation : [Sensors_20.O_24_Cart_Next == true && ...
        | status3 == true]
    CartToProcessing.DetectionofCartNumberinStation -> CartToProcessing.CartPassesNextStation : [Sensors_20.O_24_Cart_Next == false && ...
        | status5 == true]
    CartToProcessing.CartGetsNearNextStation -> CartToProcessing.DetectionofCartNumberinStation : [AS_i_90.A_93_TestCartID == 0 && ...
        | status4 == true]
    CartToProcessing.CartPassesNextStation -> CartToProcessing.CartArrivesinNextStation : [Sensors_20.O_25_Cart_Stat == true && ...
        | status6 == true]
    CartToProcessing.StartsProcess -> CartToProcessing.CartStartsMoving [order 1] : [Sensors_20.O_24_Cart_Stat == false && ...
        |  status2 == true]
    CartToProcessing.InitialCondition -> CartToProcessing.StartsProcess : [Control_20.C_25_Request == true && ...
        |  status == true]
    CartToProcessing.CartArrivesinNextStation -> (junction 1033)
    CartToProcessing.StartsProcess -> CartToProcessing.T1 [order 2] : [after(2, sec)]
    (junction 1033) -> CartToProcessing.T3 [order 2] : [after(3,sec)]
    (junction 1033) -> CartToProcessing.T2 [order 1] : [after(2,sec)]
  state Handling_1_Cart_to_Processing
    state InitialCondition
      entry:
      status = false;
      during:
      Sensors_90.O_91_Key_Pos;
      Sensors_90.O_91_Start;
      Controls_90.C_95_Start;
      AS_i_90.A_94_CRoute_In;
      if
      status = true;
      else
      status = false;
      end
    state VarDeclaration_90
      entry:
      %AS_i_90
      AS_i_90.A_94_Request;
      AS_i_90.A_94_No_Cart;
      AS_i_90.A_94_Cart_Full;
      AS_i_90.A_94_CRoute_Out;
      AS_i_90.A_93_ProcCartID;
      AS_i_90.A_94_Cart_Stat;
      AS_i_90.A_94_Cart_Next;
      AS_i_90.A_94_Optic;
      AS_i_90.A_94_Count;
      AS_i_90.A_94_Pist_Bck;
      AS_i_90.A_94_Release_FB;
      AS_i_90.A_94_CRoute_In;
      %Control_90
      Control_90.C_95_Initialization;
      Control_90.C_95_PD_Proc;
      Control_90.C_95_PD_Cart;
      Control_90.C_92_Profibus;
      Control_90.C_95_Start
      Control_90.C_95_Cart2Del;
      Control_90.C_95_Del2Cart;
      %Actuators_90
      Actuators_90.F_92_Claw_2_Cart;
      Actuators_90.F_92_Claw_2_Del;
      Actuators_90.F_92_Claw_Down;
      Actuators_90.F_92_Close_Claw;
      Actuators_90.F_93_Led_Start;
      Actuators_90.F_93_Led_Reset;
      Actuators_90.F_93_Led_Extra1;
      Actuators_90.F_93_Led_Extra2;
      Actuators_90.F_93_Panel_O4;
      Actuators_90.F_93_Panel_O5;
      Actuators_90.F_93_Panel_O6;
      Actuators_90.F_93_Panel_O7;
      %Sensors_90
      Sensors_90.O_90_Part_Reserve;
      Sensors_90.O_90_Claw_Del;
      Sensors_90.O_90_Claw_Cart;
      Sensors_90.O_90_Claw_Reserve;
      Sensors_90.O_90_Claw_Low;
      Sensors_90.O_90_Claw_High;
      Sensors_90.O_90_Part_in_Claw;
      Sensors_90.O_91_Start;
      Sensors_90.O_91_Stop;
      Sensors_90.O_91_Key_Pos;
      Sensors_90.O_91_Reset;
      Sensors_90.O_91_Panel_I4;
      Sensors_90.O_91_Panel_I5;
      Sensors_90.O_91_Panel_I6;
      Sensors_90.O_91_Panel_I7;
    (default) -> Handling_1_Cart_to_Processing.InitialCondition
  (default) -> VarDeclaration_100
  VarDeclaration_40 -> VarDeclaration_30
  VarDeclaration_30 -> VarDeclaration_20
  VarDeclaration_100 -> VarDeclaration_90
  VarDeclaration_90 -> VarDeclaration_80
  VarDeclaration_80 -> VarDeclaration_70
  VarDeclaration_60 -> VarDeclaration_50
  VarDeclaration_50 -> VarDeclaration_40
  VarDeclaration_70 -> VarDeclaration_60
  VarDeclaration_20 -> Start
  Start -> CartToTesting : [Control_20.C_24_Request == true]
  CartToTesting -> (junction 1047) : [Control_20.C_24_CartDel == true]
  (junction 1047) -> (junction 1049)
  Distribution_Single -> (junction 829) : [Control_80.C_85_Part_Del == true]
  (junction 829) -> (junction 826)
  (junction 729) -> (junction 999)
  (junction 999) -> Distribution_Single
  (junction 726) -> (junction 729) [order 1] : [Control_80.C_85_Single == true]
  (junction 993) -> (junction 999) : [Control_70.C_75_RQ_Wrong == true]
  Identified_Delivery -> (junction 968) : [Control_70.C_75_Part_Del == true]
  (junction 832) -> Identified_Delivery
  (junction 968) -> (junction 971)
  (junction 831) -> (junction 832) [order 2] : [Control_70.C_75_Identified == true]
  (junction 1049) -> (junction 726)
  (junction 726) -> (junction 996) [order 3] : [Control_80.C_85_Continuous == true]
  (junction 996) -> Distribution_Continuous
  (junction 726) -> (junction 732) [order 2] : [Control_80.C_85_Counted == true]
  (junction 992) -> (junction 996) [order 1] : [Control_70.C_75_RQ_Wrong == true]
  Distribution_Continuous -> (junction 826) : [Control_80.C_85_Part_Del == true]
  (junction 826) -> (junction 831)
  (junction 971) -> (junction 1044)
  (junction 827) -> (junction 826)
  (junction 831) -> (junction 833) [order 1] : [Control_70.C_75_Requested == true]
  (junction 967) -> (junction 971)
  (junction 1044) -> CartToProcessing : [Control_20.C_25_Request == true]
  (junction 833) -> Requested_Delivery
  Requested_Delivery -> (junction 967) [order 1] : [Control_70.C_75_Part_Del == true]
  (junction 732) -> (junction 987)
  (junction 987) -> Distribution_Counted
  (junction 982) -> (junction 987) [order 1] : [Control_70.C_75_RQ_Wrong == true]
  Distribution_Counted -> (junction 827) : [Control_80.C_85_Part_Del == true]
  Requested_Delivery -> (junction 965) [order 2] : [Control_70.C_75_RQ_Wrong == true]
  (junction 965) -> (junction 982)
  (junction 992) -> (junction 993) [order 2]
  (junction 982) -> (junction 992) [order 2]
  CartToProcessing -> Handling_1_Cart_to_Processing : [Control_20.C_25_CartDel == true]
  data: Control_80 input Bus: B_Control_80; Actuators_80 input Bus: B_Actuators_80; Sensors_80 input Bus: B_Sensors_80; AS_i_70 input Bus: B_AS_i_70; Control_70 input Bus: B_Control_70; Actuators_70 input Bus: B_Actuators_70; Sensors_70 input Bus: B_Sensors_70; C_82_Profibus local; C_83_RQ_Parts local; C_85_Continuous local; C_85_Counted local; C_85_Initialization local; C_85_Part_Del local; C_85_Single local; C_85_Start local; F_82_Arm_2_Del local; F_82_Arm_2_Mag local; F_82_Pist_Adv local; F_82_Suction_Off local; F_82_Suction_On local; F_83_Led_Extra1 local; F_83_Led_Extra2 local; F_83_Led_Reset local; F_83_Led_Start local; F_83_Panel_O4 local; F_83_Panel_O5 local; F_83_Panel_O6 local; F_83_Panel_O7 local; O_80_Arm_Del local; O_80_Arm_Mag local; O_80_Mag_Empty local; O_80_Mag_Full local; O_80_Part_Stuck local; O_80_Pist_Back local; O_80_Pist_Fwd local; O_81_Key_Pos local; O_81_Panel_I4 local; O_81_Panel_I5 local; O_81_Panel_I6 local; O_81_Panel_I7 local; O_81_Reset local; O_81_Start local; O_81_Stop local; C_75_ID_Delivery1 local; C_75_ID_Delivery2 local; C_75_Identified local; C_75_Identified80 local; C_75_Initialization local; C_75_Part_Del local; C_75_RQ_Delivery1 local; C_75_RQ_Delivery2 local; C_75_RQ_Part_Del local; C_75_RQ_Wrong local; C_75_Requested local; C_75_Requested80 local; F_72_Air_On local; F_72_Eject_Part local; F_72_Elev_Down local; F_72_Elev_Up local; F_73_Led_Extra1 local; F_73_Led_Extra2 local; F_73_Led_Reset local; F_73_Led_Start local; F_73_Panel_O4 local; F_73_Panel_O5 local; F_73_Panel_O6 local; F_73_Panel_O7 local; O_70_Elev_High local; O_70_Elev_Low local; O_70_Pist_Back local; O_70_SInductive local; O_70_SPart local; O_70_SPart_Height local; O_70_SStation local; O_71_Key_Pos local; O_71_Panel_I4 local; O_71_Panel_I5 local; O_71_Panel_I6 local; O_71_Panel_I7 local; O_71_Reset local; O_71_Start local; O_71_Stop local; A_73_TestCartID local; A_74_CRoute_In local; A_74_CRoute_In80 local; A_74_CRoute_Out local; A_74_Cart_Full local; A_74_Cart_Next local; A_74_Cart_Stat local; A_74_Count local; A_74_No_Cart local; A_74_Optic local; A_74_Pist_Bck local; A_74_Release_FB local; A_74_Request local; C_72_Profibus local; AS_i_30 input Bus: B_AS_i_30; AS_i_50 input Bus: B_AS_i_50; AS_i_90 input Bus: B_AS_i_90; Actuators_100 input Bus: B_Actuators_100; Actuators_20 input Bus: B_Actuators_20; Actuators_30 input Bus: B_Actuators_30; Actuators_50 input Bus: B_Actuators_50; Actuators_60 input Bus: B_Actuators_60; Actuators_90 input Bus: B_Actuators_90; Control_100 input Bus: B_Control_100; Control_20 input Bus: B_Control_20; Control_30 input Bus: B_Control_30; Control_50 input Bus: B_Control_50; Control_60 input Bus: B_Control_60; Control_90 input Bus: B_Control_90; Sensors_100 input Bus: B_Sensors_100; Sensors_20 input Bus: B_Sensors_20; Sensors_30 input Bus: B_Sensors_30; Sensors_50 input Bus: B_Sensors_50; Sensors_60 input Bus: B_Sensors_60; Sensors_90 input Bus: B_Sensors_90; A_32_RoboCartID local; A_34_CRoute_In local; A_34_CRoute_Out local; A_34_Cart_Full local; A_34_Cart_Next local; A_34_Cart_Stat local; A_34_Count local; A_34_No_Cart local; A_34_Optic local; A_34_Pist_Bck local; A_34_Release_FB local; A_34_Request local; A_53_SortCartID local; A_54_CRoute_In local; A_54_CRoute_Out local; A_54_Cart_Full local; A_54_Cart_Next local; A_54_Cart_Stat local; A_54_Count local; A_54_No_Cart local; A_54_Optic local; A_54_Pist_Bck local; A_54_Release_FB local; A_54_Request local; A_93_ProcCartID local; A_94_CRoute_In local; A_94_CRoute_Out local; A_94_Cart_Full local; A_94_Cart_Next local; A_94_Cart_Stat local; A_94_Count local; A_94_No_Cart local; A_94_Optic local; A_94_Pist_Bck local; A_94_Release_FB local; A_94_Request local; C_102_Profibus local; C_103_RQ_Turns local; C_105_Initialization local; C_105_Part_ready local; C_105_Rotation local; C_105_Start local; C_105_Test local; C_105_TestDrill local; C_105_Test_Fail local; C_105_Test_Ok local; C_24_CRoute_In local; C_24_CRoute_Out local; C_24_CartDel local; C_24_Request local; C_25_CRoute_In local; C_25_CRoute_Out local; C_25_CartDel local; C_25_Request local; C_26_CRoute_In local; C_26_CRoute_Out local; C_26_CartDel local; C_26_Request local; C_27_CRoute_In local; C_27_CRoute_Out local; C_27_CartDel local; C_27_Request local; C_28_CRoute_In local; C_28_CRoute_Out local; C_28_CartDel local; C_28_Request local; C_29_CRoute_In local; C_29_CRoute_Out local; C_29_CartDel local; C_29_Request local; C_30_Robot1 local; C_30_Robot2 local; C_35_Part_Del local; C_52_Profibus local; C_55_Cart2Del local; C_55_Initialization local; C_55_PD_Sort local; C_55_Start local; C_62_Profibus local; C_65_BRS_Output local; C_65_BSR_Output local; C_65_ID_1 local; C_65_ID_2 local; C_65_Initialization local; C_65_RBS_Output local; C_65_RSB_Output local; C_65_SBR_Output local; C_65_SRB_Output local; C_92_Profibus local; C_95_Cart2Del local; C_95_Del2Cart local; C_95_Initialization local; C_95_PD_Cart local; C_95_PD_Proc local; C_95_Start local; F_102_Drill_Down local; F_102_Drill_On local; F_102_Drill_Pin local; F_102_Drill_Up local; F_102_RT_On local; F_102_Test_Pin local; F_103_Led_Extra1 local; F_103_Led_Extra2 local; F_103_Led_Reset local; F_103_Led_Start local; F_103_Panel_O4 local; F_103_Panel_O5 local; F_103_Panel_O6 local; F_103_Panel_O7 local; F_22_Led_Off local; F_22_Led_On local; F_24_Release_FB local; F_25_Release_FB local; F_26_Release_FB local; F_27_Release_FB local; F_28_Release_FB local; F_29_Release_FB local; F_33_Cover_Cyl local; F_33_Led_Extra1 local; F_33_Led_Extra2 local; F_33_Led_Reset local; F_33_Led_Start local; F_33_Spring_Cyl local; F_52_Claw_2_Cart local; F_52_Claw_2_Del local; F_52_Claw_Down local; F_52_Close_Claw local; F_53_Led_Extra1 local; F_53_Led_Extra2 local; F_53_Led_Reset local; F_53_Led_Start local; F_53_Panel_O4 local; F_53_Panel_O5 local; F_53_Panel_O6 local; F_53_Panel_O7 local; F_62_Conveyor local; F_62_Identify local; F_62_P1 local; F_62_P2 local; F_63_Led_Extra1 local; F_63_Led_Extra2 local; F_63_Led_Reset local; F_63_Led_Start local; F_63_Panel_O4 local; F_63_Panel_O5 local; F_63_Panel_O6 local; F_63_Panel_O7 local; F_92_Claw_2_Cart local; F_92_Claw_2_Del local; F_92_Claw_Down local; F_92_Close_Claw local; F_93_Led_Extra1 local; F_93_Led_Extra2 local; F_93_Led_Reset local; F_93_Led_Start local; F_93_Panel_O4 local; F_93_Panel_O5 local; F_93_Panel_O6 local; F_93_Panel_O7 local; O_100_PDrill_Pos local; O_100_PInit_Pos local; O_100_PTest_Ok local; O_100_PTest_Pos local; O_100_RT_Sensor local; O_100_SDrill_High local; O_100_SDrill_Low local; O_101_Key_Pos local; O_101_Panel_I4 local; O_101_Panel_I5 local; O_101_Panel_I6 local; O_101_Panel_I7 local; O_101_Reset local; O_101_Start local; O_101_Stop local; O_20_Controler_On local; O_20_Off local; O_20_On local; O_24_Cart_Next local; O_24_Cart_Stat local; O_24_Count local; O_24_Optic local; O_24_Pist_Bck local; O_25_Cart_Next local; O_25_Cart_Stat local; O_25_Count local; O_25_Optic local; O_25_Pist_Back local; O_26_Cart_Next local; O_26_Cart_Stat local; O_26_Count local; O_26_Optic local; O_26_Pist_Back local; O_27_Cart_Next local; O_27_Cart_Stat local; O_27_Count local; O_27_Optic local; O_27_Pist_Back local; O_28_Cart_Next local; O_28_Cart_Stat local; O_28_Count local; O_28_Optic local; O_28_Pist_Back local; O_29_Cart_Next local; O_29_Cart_Stat local; O_29_Count local; O_29_Optic local; O_29_Pist_Back local; O_31_Orientation local; O_31_Part_in_Claw local; O_31_Reset local; O_31_Start local; O_31_Stop local; O_32_CoMag_Empty local; O_32_Co_Cyl_Bck local; O_32_Co_Cyl_Fwd local; O_32_Co_PickUp local; O_32_Sp_Cyl_Bck local; O_32_Sp_Cyl_Fwd local; O_32_Sp_PickUp local; O_50_Claw_Cart local; O_50_Claw_Del local; O_50_Claw_High local; O_50_Claw_Low local; O_50_Claw_Reserve local; O_50_Part_Reserve local; O_50_Part_in_Claw local; O_51_Key_Pos local; O_51_Panel_I4 local; O_51_Panel_I5 local; O_51_Panel_I6 local; O_51_Panel_I7 local; O_51_Reset local; O_51_Start local; O_51_Stop local; O_60_Part_Pass local; O_60_SL1_Bck local; O_60_SL1_Fwd local; O_60_SL2_Bck local; O_60_SL2_Fwd local; O_60_SPart local; O_60_SPhoto local; O_60_Slnd local; O_61_Key_Pos local; O_61_Panel_I4 local; O_61_Panel_I5 local; O_61_Panel_I6 local; O_61_Panel_I7 local; O_61_Reset local; O_61_Start local; O_61_Stop local; O_90_Claw_Cart local; O_90_Claw_Del local; O_90_Claw_High local; O_90_Claw_Low local; O_90_Claw_Reserve local; O_90_Part_Reserve local; O_90_Part_in_Claw local; O_91_Key_Pos local; O_91_Panel_I4 local; O_91_Panel_I5 local; O_91_Panel_I6 local; O_91_Panel_I7 local; O_91_Reset local; O_91_Start local; O_91_Stop local; F_22_Conveyor local; status6 local; status local; status2 local; status3 local; status4 local; status5 local; status7 local; status1 local; status10 local; status11 local; status12 local; status13 local; status9 local; status8 local; status14 local; LoopDistCont local; Control_40 input Bus: B_Control_40; AS_i_40 input Bus: B_AS_i_40; Actuators_40 input Bus: B_Actuators_40; Sensors_40 input Bus: B_Sensors_40; A_44_CRoute_In local; A_44_CRoute_Out local; A_44_Cart_Full local; A_44_Cart_Next local; A_44_Cart_Stat local; A_44_Count local; A_44_No_Cart local; A_44_Optic local; A_44_Pist_Bck local; A_44_Release_FB local; A_44_Request local; C_42_Profibus local; C_45_Initialization local; C_45_RetrievePart local; C_45_Start local; C_45_StorePart local; F_43_Led_Extra1 local; F_43_Led_Extra2 local; F_43_Led_Reset local; F_43_Led_Start local; F_43_Panel_O4 local; F_43_Panel_O5 local; F_43_Panel_O6 local; F_43_Panel_O7 local; O_41_Key_Pos local; O_41_Panel_I4 local; O_41_Panel_I5 local; O_41_Panel_I6 local; O_41_Panel_I7 local; O_41_Reset local; O_41_Start local; O_41_Stop local; C_86_Mag_Parts local; A_43_StorCartID local; C_85_Part_Mag local; C_87_RQ_MParts local; MetalicPart local; Part_Equal local; Part_Different local; status15 local; status16 local; status18 local; status17 local; status19 local
